simulink model "jumeau_banc_rw"  (R2025b)
settings: Solver=ode23t  StartTime=0.0  StopTime=20  MaxStep=1e-3  RelTol=1e-4
PostLoadFcn:
  | d = fileparts(get_param('jumeau_banc_rw', 'FileName')); addpath(fullfile(d, 'geometrie'), fullfile(d, 'liaison'), fullfile(d, 'pilotage')); clear d
StartFcn:
  | % Jumeau Webots : au lancement, MATLAB envoie les paramètres du Model Workspace à Webots, qui remet le banc en
  | % position de départ, puis ouvre la liaison de télémétrie et la liaison de commande (liaison/pont_banc.m).
  | if strcmp(get_param('jumeau_banc_rw/Procédé', 'LabelModeActiveChoice'), 'Webots')
  |     pont_banc('ouvrir', getVariable(get_param('jumeau_banc_rw', 'ModelWorkspace'), 'config_jumeau'));
  | end
  | pilotage_banc('depart');   % interface de pilotage : nouveau lancement
StopFcn:
  | pont_banc('fermer');
  | pilotage_banc('fin');
model workspace (MATLAB code in the model file):
  | %% Jumeau numérique du banc de stabilisation à 4 roues de réaction (version 3) : paramètres
  | % Ce code est enregistré dans le modèle (Model Explorer > jumeau_banc_rw > Model Workspace).
  | % Origine : (CAO) CAO du banc version 3, (M) mesuré sur le matériel, (F) fiche technique, (Fw) firmware,
  | % (H) hypothèse à mesurer sur le banc. Masses et inerties des pièces : dans chaque bloc de pièce.
  | 
  | %% Montage de l'essai
  | pivot_mm = 25;              % position du pivot de tangage sur le corps : 25, 24, 16, 8, 0, -8 mm (25 : banc équilibré, rangée +24 et paliers remontés de 1 mm)
  | blocage_roulis = 0;         % goupille de blocage : 1 = axe bloqué à 0°, 0 = axe libre
  | blocage_tangage = 0;
  | angle0_roulis_deg = 2;      % position de départ (mise à 0 si l'axe est bloqué)
  | angle0_tangage_deg = -1;
  | g = 9.81;                   % m/s²
  | 
  | %% Pupitre : pilotage manuel des 4 ESC
  | essai_t = 1;                % s, instant de l'échelon d'essai ajouté aux curseurs
  | essai_echelon_us = [0 0 0 0];   % µs, échelon d'essai sur chaque ESC (0 : aucun)
  | 
  | %% Alimentation des ESC
  | V_alim = 12;                % V, alimentation de labo (H : tension réglée)
  | 
  | %% ESC Brushless 30A bidirectionnels (x4)
  | f_trame_esc = 50;           % Hz, une impulsion toutes les 20 ms (Fw : LEDC 50 Hz)
  | imp_neutre = 1500;          % µs, neutre (testé sur le banc)
  | imp_min = 1000;             % µs (Fw)
  | imp_max = 2000;             % µs (Fw)
  | zone_morte_us = 0;          % µs autour du neutre (H)
  | tau_esc = 2e-3;             % s, temps de réponse de l'ESC (H)
  | armement_actif = 1;         % 1 : l'ESC ne pilote le moteur qu'après t_armement au neutre
  | t_armement = 1;             % s (H)
  | fenetre_armement_us = 25;   % µs, écart au neutre accepté pendant l'armement (H)
  | sens_moteurs = [1 1 1 1];   % +1 : au-dessus du neutre, la roue tourne dans le sens +axe (vers l'extérieur) (H : ordre des phases)
  | 
  | %% Moteurs A2212 1400 KV (x4), modèle équivalent continu
  | KV = 1400;                  % tr/min/V (F)
  | Ke = 60/(2*pi*KV);          % V.s/rad
  | Kt = Ke;                    % N.m/A
  | R_moteur = 0.08;            % ohm (H)
  | L_moteur = 30e-6;           % H (H)
  | f_roue = 5e-6;              % N.m.s/rad, frottement visqueux des roulements du moteur (H)
  | 
  | %% Cardan
  | butee_deg = 20;             % débattement de chaque axe (CAO)
  | k_butee = 20;               % N.m/rad, contact goupille-lumière (H)
  | c_butee = 0.2;              % N.m.s/rad (H)
  | b_cardan = 1e-4;            % N.m.s/rad, frottement des roulements 625 (H)
  | k_cables = 0;               % N.m/rad, raideur des deux câbles vers la table (H)
  | 
  | %% BNO055 (mode fusion)
  | T_bno = 0.01;               % s, données de fusion à 100 Hz (F)
  | bruit_bno = 1;              % 1 : bruit de mesure, 0 : capteur parfait
  | sigma_angle_deg = 0.05;     % ° (H)
  | sigma_gyro_dps = 0.1;       % °/s (H)
  | sigma_acc = 0.02;           % m/s² (H)
  | R_montage_bno = eye(3);     % axes du capteur dans le repère du dispositif : eye(3) = remappage AXIS_MAP réglé
  |                             % (la carte est tournée de 90° dans la CAO)
  | 
  | %% Capteurs de vitesse TCRT5000 (x4) : un front à chaque rayon du disque
  | n_rayons = 4;               % rayons du disque vus par tour (CAO : disque d'origine)
  | T_tcrt = 1e-3;              % s, pas de calcul du capteur (les fronts sont datés par interpolation, comme un chronomètre en µs)
  | t_arret_tcrt = 0.2;         % s sans front : la vitesse mesurée retombe à 0 (Fw, à fixer)
  | 
  | %% Pont vers le jumeau Webots (et, plus tard, vers l'ESP32 du banc réel)
  | T_pont = 0.01;              % s, une trame de commande et une trame de télémétrie toutes les 10 ms
  | 
  | %% Essai : maintien au départ et perturbation
  | t_lacher = 2;                % s, le dispositif est tenu à la main à sa position de départ jusqu'à cet instant (0 : libre dès le départ)
  | k_main = 5;                  % N.m/rad, raideur de la main qui tient le dispositif
  | c_main = 0.3;                % N.m.s/rad, son amortissement
  | perturbation_t = 7;          % s, instant de la poussée d'essai
  | perturbation_duree = 0.2;    % s
  | perturbation_couple = [0.02 0.02];   % N.m, couple de la poussée sur [roulis tangage], programmée (0 : aucune ; l'interface de pilotage en ajoute)
  | 
  | %% Grandeurs dérivées
  | assert(any(pivot_mm == [25 24 16 8 0 -8]), 'pivot_mm : 25, 24, 16, 8, 0, -8');
  | q0_deg = [angle0_roulis_deg angle0_tangage_deg] .* ([blocage_roulis blocage_tangage] == 0);
  | config_jumeau = [pivot_mm; blocage_roulis; blocage_tangage; q0_deg(:); V_alim; f_trame_esc; imp_neutre; imp_min; imp_max; ...
  |     zone_morte_us; tau_esc; armement_actif; t_armement; fenetre_armement_us; sens_moteurs(:); Ke; Kt; R_moteur; L_moteur; ...
  |     f_roue; butee_deg; k_butee; c_butee; b_cardan; k_cables; g; T_bno; bruit_bno; sigma_angle_deg; sigma_gyro_dps; ...
  |     sigma_acc; n_rayons; t_arret_tcrt; T_tcrt; R_montage_bno(:); T_pont; t_lacher; k_main; c_main];   % 51 valeurs envoyées au jumeau Webots au lancement
  | 
  | %% Commande bas niveau : une boucle de vitesse par roue, avec observateur CFO (méthode du TP2, ramenée à la vitesse)
  | J_roue = 1.562e-4;          % kg.m², inertie d'une roue autour de son axe : disque, vis, cloche du moteur (CAO)
  | T_cbn = 1/f_trame_esc;      % s, période de calcul de la commande : celle des ESC, qui ne lisent qu'une impulsion toutes les 20 ms
  | wc_roue = [10 10 10 10];    % rad/s, rapidité du suivi de vitesse de chaque roue (pôle de l'erreur en -wc)
  | wo_roue = [5 5 5 5];        % rad/s, rapidité du CFO de chaque roue (pôles en -wo et -4 wo) ; au-delà de 10, il devient instable à 20 ms
  | imp_cmd_min = 1375;         % µs, limites des impulsions commandées : vitesse conseillée des disques, 3 900 tr/min
  | imp_cmd_max = 1625;         % µs
  | w_aveugle = 45;             % rad/s, en dessous (vitesse du modèle), le TCRT5000 voit mal la roue : le CFO ne se corrige plus sur la mesure
  | 
  | %% Consigne d'essai des roues : ajoutée à la consigne qui vient de la conversion (0 tant qu'elle est vide)
  | essai_roue_t1 = 2;                  % s, départ vers le premier palier
  | essai_roue_vitesse1 = [0 0 0 0];  % rad/s, premier palier de chaque roue (0 : la roue reste à l'arrêt)
  | essai_roue_t2 = 6;                  % s, départ vers le second palier
  | essai_roue_vitesse2 = [0 0 0 0];    % rad/s, second palier de chaque roue
  | essai_roue_acc = 300;               % rad/s², pente des rampes entre les paliers
  | 
  | %% Commande bas niveau : grandeurs calculées
  | % modèle local d'une roue : d(omega)/dt = -a1 omega + a0 V + d
  | a0_roue = Kt/(R_moteur*J_roue) * [1 1 1 1];                % rad/s² par volt
  | a1_roue = (Kt*Ke/R_moteur + f_roue)/J_roue * [1 1 1 1];    % 1/s
  | K_roue = wc_roue - a1_roue;                                % retour d'état : erreur en -(a1 + K) = -wc
  | l1_roue = 5*wo_roue;                                       % CFO
  | lambda_roue = 4/5*wo_roue;
  | 
  | %% Référence : angles demandés au dispositif, en polynômes de degré 5 entre deux paliers
  | ref_t = [2 12];              % s, instant de départ vers chaque palier
  | ref_roulis_deg = [0 5];      % °, roulis demandé à chaque palier
  | ref_tangage_deg = [0 0];     % °, tangage demandé à chaque palier
  | ref_duree = 1.5;             % s, durée du passage d'un palier au suivant
  | 
  | %% Commande haut niveau : une boucle par axe [roulis tangage], placement de pôles basé sur l'observateur CFO (TP2)
  | T_chn = T_cbn;               % s, période de calcul : celle de la commande bas niveau et des ESC
  | t_depart = t_lacher;         % s, mise en marche de la commande : au moment où la main lâche le dispositif
  | wc_axe = [4 4];              % rad/s, rapidité du suivi d'angle de chaque axe
  | xi_axe = [1 1];              % amortissement
  | wo_axe = [3 3];              % rad/s, rapidité du CFO de chaque axe (pôles en -wo et -4 wo, double) ; au-delà de 4, le couple s'agite
  | desat_active = 0;            % 1 : la référence est décalée pour ramener les roues vers leur vitesse de repos
  | T_desat = 5;                 % s, constante de temps de ce retour
  | desat_max_deg = 15;          % °, décalage maximal de la référence
  | 
  | %% Conversion : couples des deux axes vers les 4 roues
  | w_repos = 200;               % rad/s, vitesse de repos des 4 roues : elles tournent toujours, le TCRT5000 les voit toujours
  | t_roues = t_armement + 0.2;  % s, mise en rotation des roues, une fois les ESC armés
  | acc_roue_max = 300;          % rad/s², accélération maximale demandée à une roue
  | w_roue_min = 60;             % rad/s, vitesses limites demandées à une roue
  | w_roue_max = 400;            % rad/s (disques : 3 900 tr/min conseillés, soit 408 rad/s)
  | 
  | %% Masses et inerties utilisées par la commande (CAO du banc version 3)
  | m_disp = 1.2615;             % kg, dispositif et ses 4 roues
  | zG_disp = 24.977e-3;         % m, hauteur de son centre de masse sur le corps (le pivot est à pivot_mm)
  | Ixx_disp_24 = 8.2684e-3;     % kg.m², inertie du dispositif autour du roulis, pivot à +24 mm
  | Iyy_disp_24 = 8.2786e-3;     % kg.m², autour du tangage, pivot à +24 mm
  | m_croix = 0.0755;            % kg, croisillon et paliers (ne tournent qu'en roulis)
  | zG_croix = 0.257e-3;         % m, hauteur de leur centre de masse au-dessus de l'axe de roulis
  | Ixx_croix = 2.073e-4;        % kg.m²
  | 
  | %% Commande haut niveau et conversion : grandeurs calculées
  | % modèle local d'un axe : d²(theta)/dt² = -a1 d(theta)/dt + a0 C + d, avec C le couple demandé aux roues
  | hz = zG_disp - pivot_mm/1000;                                    % m, centre de masse du dispositif au-dessus du pivot
  | I_axe = [Ixx_disp_24 + Ixx_croix, Iyy_disp_24] + m_disp*(hz^2 - (zG_disp - 0.024)^2) - 2*J_roue;   % kg.m²
  | mgh_axe = g*[m_disp*hz + m_croix*zG_croix, m_disp*hz];           % N.m/rad, couple de pesanteur par radian d'inclinaison
  | a0_axe = 1./I_axe;                                               % rad/s² par N.m
  | a1_axe = b_cardan./I_axe;                                        % 1/s
  | k1_axe = wc_axe.^2;                                              % retour d'état : s² + 2 xi wc s + wc²
  | k2_axe = 2*xi_axe.*wc_axe - a1_axe;
  | l1_axe = 9*wo_axe;                                               % CFO du TP2
  | l2_axe = 12*wo_axe.^2;
  | lambda_axe = 4/3*wo_axe;
  | C_max = 2*J_roue*cosd(45)*acc_roue_max;                          % N.m, couple maximal demandé sur un axe
  | k_desat = desat_active.*sign(mgh_axe + (mgh_axe == 0))./(max(abs(mgh_axe), 1e-3)*T_desat);            % rad par N.m.s
  | sx_roues = [1 -1 -1 1];                                          % signe de cos(45°, 135°, 225°, 315°) : part de chaque roue sur le roulis
  | sy_roues = [1 1 -1 -1];                                          % signe de sin : part sur le tangage
  | M_conv = -[sx_roues(:) sy_roues(:)]/(4*J_roue*cosd(45));         % accélération des 4 roues pour un couple [roulis; tangage]
  | 
  | %% Perception : des mesures à l'état du banc
  | T_perception = T_bno;        % s, période de calcul : celle du BNO055
  | tau_desequilibre = 2;        % s, constante de temps du filtre du couple extérieur et du déséquilibre
  | 
  | %% Pilotage par l'interface (pilotage/pilote_banc.m)
  | manche_max_deg = 15;         % °, limite de sécurité de l'inclinaison demandée par le manche (l'interface règle l'amplitude)
  | w_manche = 3;                % rad/s, rapidité avec laquelle la référence rejoint le manche (second ordre critique)
  | T_affichage = 0.1;           % s, rafraîchissement de l'interface
undefined symbols (not defined in the file): DiscIntNeverNeededParam, X, Y, Z
libraries: sm_lib x256, nesl_utility x24, simulink x7
(part 4 of 8)

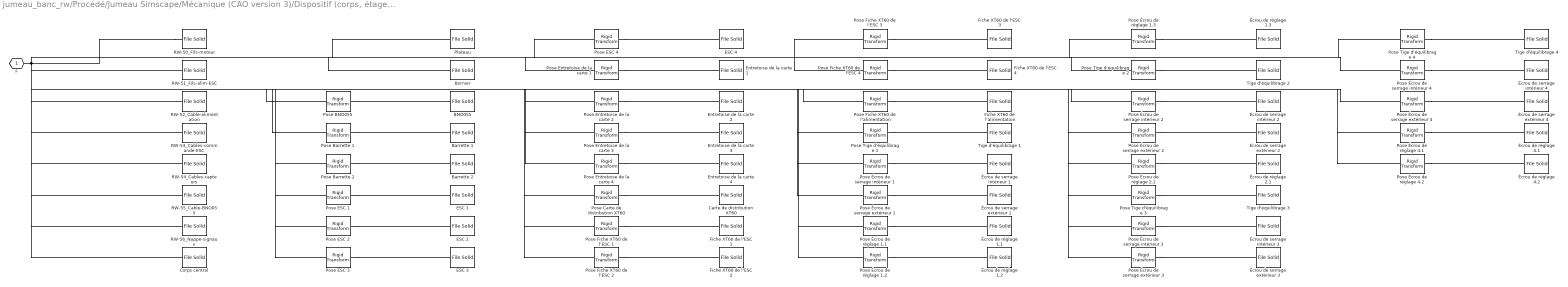
== system jumeau_banc_rw/Procédé/Jumeau Simscape/Mécanique (CAO version 3)/Dispositif (corps, étage, électronique, câblage) ==
  BNO055 : sm_lib/Body Elements/File Solid  Description=|  ExtGeomFileName=RW-32_BNO055.stl  UnitType=Custom  ExtGeomFileUnits=mm  StepReaderType=HEX  ExportConvexHullGeometry=off  InertiaType=Custom  BasedOnType=DensityFromFile  Density=1000  DensityUnits=kg/m^3  Mass=0.003  MassUnits=kg  CenterOfMass=[-2.1467412e-19 -0.0018514253 0.0013309763]  CenterOfMassUnits=m  MomentsOfInertia=[1.3564844e-07 1.7232429e-07 2.8762159e-07]  MomentsOfInertiaUnits=kg*m^2  ProductsOfInertia=[1.2064608e-08 -8.9985138e-25 -1.6417474e-24]  ProductsOfInertiaUnits=kg*m^2  GraphicType=FromGeometry  MarkerShape=Sphere  MarkerSize=10  GraphicVisPropType=SimpleVisualProperties  GraphicDiffuseColor=[0.173 0.627 0.173]  GraphicOpacity=1  GraphicSpecularColor=[0.5 0.5 0.5 1.0]  GraphicAmbientColor=[0.15 0.15 0.15 1.0]  GraphicEmissiveColor=[0.0 0.0 0.0 1.0]  GraphicShininess=75  DoExposeReferenceFrame=on  SerializedFrames=<Frames/>
      | Pièce CAO : BNO055 (RW-32_BNO055)
      | Masse 3.00 g : GY-BNO055, fiche, 3 g répartis sur le volume de la CAO.
      | Centre de masse et inertie : calculés sur la géométrie de la CAO.
  Barrette 1 : sm_lib/Body Elements/File Solid  Description=|  ExtGeomFileName=RW-36_Barrette-1x15.stl  UnitType=Custom  ExtGeomFileUnits=mm  StepReaderType=HEX  ExportConvexHullGeometry=off  InertiaType=Custom  BasedOnType=DensityFromFile  Density=1000  DensityUnits=kg/m^3  Mass=0.001  MassUnits=kg  CenterOfMass=[9.3534391e-19 3.3043458e-22 0.00027234952]  CenterOfMassUnits=m  MomentsOfInertia=[1.4288155e-08 1.347296e-07 1.2118031e-07]  MomentsOfInertiaUnits=kg*m^2  ProductsOfInertia=[-1.6381112e-26 2.6393535e-24 -2.0442735e-26]  ProductsOfInertiaUnits=kg*m^2  GraphicType=FromGeometry  MarkerShape=Sphere  MarkerSize=10  GraphicVisPropType=SimpleVisualProperties  GraphicDiffuseColor=[0.133 0.133 0.133]  GraphicOpacity=1  GraphicSpecularColor=[0.5 0.5 0.5 1.0]  GraphicAmbientColor=[0.15 0.15 0.15 1.0]  GraphicEmissiveColor=[0.0 0.0 0.0 1.0]  GraphicShininess=75  DoExposeReferenceFrame=on  SerializedFrames=<Frames/>
      | Pièce CAO : Barrette 1 (RW-36_Barrette-1x15)
      | Masse 1.00 g : barrette 1 × 15, estimée, 1 g répartis sur le volume de la CAO.
      | Centre de masse et inertie : calculés sur la géométrie de la CAO.
  Barrette 2 : sm_lib/Body Elements/File Solid  Description=|  ExtGeomFileName=RW-36_Barrette-1x15.stl  UnitType=Custom  ExtGeomFileUnits=mm  StepReaderType=HEX  ExportConvexHullGeometry=off  InertiaType=Custom  BasedOnType=DensityFromFile  Density=1000  DensityUnits=kg/m^3  Mass=0.001  MassUnits=kg  CenterOfMass=[9.3534391e-19 3.3043458e-22 0.00027234952]  CenterOfMassUnits=m  MomentsOfInertia=[1.4288155e-08 1.347296e-07 1.2118031e-07]  MomentsOfInertiaUnits=kg*m^2  ProductsOfInertia=[-1.6381112e-26 2.6393535e-24 -2.0442735e-26]  ProductsOfInertiaUnits=kg*m^2  GraphicType=FromGeometry  MarkerShape=Sphere  MarkerSize=10  GraphicVisPropType=SimpleVisualProperties  GraphicDiffuseColor=[0.133 0.133 0.133]  GraphicOpacity=1  GraphicSpecularColor=[0.5 0.5 0.5 1.0]  GraphicAmbientColor=[0.15 0.15 0.15 1.0]  GraphicEmissiveColor=[0.0 0.0 0.0 1.0]  GraphicShininess=75  DoExposeReferenceFrame=on  SerializedFrames=<Frames/>
      | Pièce CAO : Barrette 2 (RW-36_Barrette-1x15)
      | Masse 1.00 g : barrette 1 × 15, estimée, 1 g répartis sur le volume de la CAO.
      | Centre de masse et inertie : calculés sur la géométrie de la CAO.
  Bornier : sm_lib/Body Elements/File Solid  Description=|  ExtGeomFileName=RW-11_Bornier.stl  UnitType=Custom  ExtGeomFileUnits=mm  StepReaderType=HEX  ExportConvexHullGeometry=off  InertiaType=Custom  BasedOnType=DensityFromFile  Density=1000  DensityUnits=kg/m^3  Mass=0.0067119926  MassUnits=kg  CenterOfMass=[-0.07837267 3.6153019e-19 0.071437544]  CenterOfMassUnits=m  MomentsOfInertia=[1.208704e-06 5.2720754e-07 1.5981936e-06]  MomentsOfInertiaUnits=kg*m^2  ProductsOfInertia=[-5.3734654e-24 7.625406e-08 1.4773525e-23]  ProductsOfInertiaUnits=kg*m^2  GraphicType=FromGeometry  MarkerShape=Sphere  MarkerSize=10  GraphicVisPropType=SimpleVisualProperties  GraphicDiffuseColor=[0.867 0.518 0.322]  GraphicOpacity=1  GraphicSpecularColor=[0.5 0.5 0.5 1.0]  GraphicAmbientColor=[0.15 0.15 0.15 1.0]  GraphicEmissiveColor=[0.0 0.0 0.0 1.0]  GraphicShininess=75  DoExposeReferenceFrame=on  SerializedFrames=<Frames/>
      | Pièce CAO : Bornier (RW-11_Bornier)
      | Masse 6.71 g : PLA imprimé, 2 parois et 15 % de remplissage (hypothèse de conception), 800 kg/m³.
      | Centre de masse et inertie : calculés sur la géométrie de la CAO.
  Carte de distribution XT60 : sm_lib/Body Elements/File Solid  Description=|  ExtGeomFileName=RW-37_Carte-XT60-1x4.stl  UnitType=Custom  ExtGeomFileUnits=mm  StepReaderType=HEX  ExportConvexHullGeometry=off  InertiaType=Custom  BasedOnType=DensityFromFile  Density=1000  DensityUnits=kg/m^3  Mass=0.05  MassUnits=kg  CenterOfMass=[0.0081065575 2.9840954e-05 0.0051344044]  CenterOfMassUnits=m  MomentsOfInertia=[3.1408208e-06 3.157647e-05 3.2701875e-05]  MomentsOfInertiaUnits=kg*m^2  ProductsOfInertia=[2.2894046e-09 -1.2849535e-07 -3.2666061e-08]  ProductsOfInertiaUnits=kg*m^2  GraphicType=FromGeometry  MarkerShape=Sphere  MarkerSize=10  GraphicVisPropType=SimpleVisualProperties  GraphicDiffuseColor=[0.169 0.169 0.169]  GraphicOpacity=1  GraphicSpecularColor=[0.5 0.5 0.5 1.0]  GraphicAmbientColor=[0.15 0.15 0.15 1.0]  GraphicEmissiveColor=[0.0 0.0 0.0 1.0]  GraphicShininess=75  DoExposeReferenceFrame=on  SerializedFrames=<Frames/>
      | Pièce CAO : Carte de distribution XT60 (RW-37_Carte-XT60-1x4)
      | Masse 50.00 g : carte de distribution XT60 1 vers 4 (Jonronfey), estimée : carte 20 g, 4 embases 20 g, entrée 10 g, soit 50 g répartis sur le volume de la CAO.
      | Centre de masse et inertie : calculés sur la géométrie de la CAO.
  Corps central : sm_lib/Body Elements/File Solid  Description=|  ExtGeomFileName=RW-01_Moyeu.stl  UnitType=Custom  ExtGeomFileUnits=mm  StepReaderType=HEX  ExportConvexHullGeometry=off  InertiaType=Custom  BasedOnType=DensityFromFile  Density=1000  DensityUnits=kg/m^3  Mass=0.14444879  MassUnits=kg  CenterOfMass=[2.4874764e-15 1.1454189e-16 0.010858243]  CenterOfMassUnits=m  MomentsOfInertia=[0.00060979177 0.00056996624 0.000928403]  MomentsOfInertiaUnits=kg*m^2  ProductsOfInertia=[1.1230228e-19 -1.1420331e-17 -1.7396122e-07]  ProductsOfInertiaUnits=kg*m^2  GraphicType=FromGeometry  MarkerShape=Sphere  MarkerSize=10  GraphicVisPropType=SimpleVisualProperties  GraphicDiffuseColor=[0.298 0.447 0.69]  GraphicOpacity=1  GraphicSpecularColor=[0.5 0.5 0.5 1.0]  GraphicAmbientColor=[0.15 0.15 0.15 1.0]  GraphicEmissiveColor=[0.0 0.0 0.0 1.0]  GraphicShininess=75  DoExposeReferenceFrame=on  SerializedFrames=<Frames/>
      | Pièce CAO : Corps central (RW-01_Moyeu)
      | Masse 144.45 g : PLA imprimé, 2 parois et 15 % de remplissage (hypothèse de conception), 800 kg/m³.
      | Centre de masse et inertie : calculés sur la géométrie de la CAO.
  ESC 1 : sm_lib/Body Elements/File Solid  Description=|  ExtGeomFileName=RW-31_ESC-30A.stl  UnitType=Custom  ExtGeomFileUnits=mm  StepReaderType=HEX  ExportConvexHullGeometry=off  InertiaType=Custom  BasedOnType=DensityFromFile  Density=1000  DensityUnits=kg/m^3  Mass=0.028  MassUnits=kg  CenterOfMass=[-2.7359067e-19 2.5376526e-20 0.007]  CenterOfMassUnits=m  MomentsOfInertia=[2.8466667e-06 1.5390667e-05 1.7322667e-05]  MomentsOfInertiaUnits=kg*m^2  ProductsOfInertia=[0 3.8857806e-24 4.4408921e-24]  ProductsOfInertiaUnits=kg*m^2  GraphicType=FromGeometry  MarkerShape=Sphere  MarkerSize=10  GraphicVisPropType=SimpleVisualProperties  GraphicDiffuseColor=[0.506 0.447 0.702]  GraphicOpacity=1  GraphicSpecularColor=[0.5 0.5 0.5 1.0]  GraphicAmbientColor=[0.15 0.15 0.15 1.0]  GraphicEmissiveColor=[0.0 0.0 0.0 1.0]  GraphicShininess=75  DoExposeReferenceFrame=on  SerializedFrames=<Frames/>
      | Pièce CAO : ESC 1 (RW-31_ESC-30A)
      | Masse 28.00 g : ESC 30 A, fiche, 28 g répartis sur l'enveloppe de 80 × 32 × 14 mm.
      | Centre de masse et inertie : calculés sur la géométrie de la CAO.
  ESC 2 : sm_lib/Body Elements/File Solid  Description=|  ExtGeomFileName=RW-31_ESC-30A.stl  UnitType=Custom  ExtGeomFileUnits=mm  StepReaderType=HEX  ExportConvexHullGeometry=off  InertiaType=Custom  BasedOnType=DensityFromFile  Density=1000  DensityUnits=kg/m^3  Mass=0.028  MassUnits=kg  CenterOfMass=[-2.7359067e-19 2.5376526e-20 0.007]  CenterOfMassUnits=m  MomentsOfInertia=[2.8466667e-06 1.5390667e-05 1.7322667e-05]  MomentsOfInertiaUnits=kg*m^2  ProductsOfInertia=[0 3.8857806e-24 4.4408921e-24]  ProductsOfInertiaUnits=kg*m^2  GraphicType=FromGeometry  MarkerShape=Sphere  MarkerSize=10  GraphicVisPropType=SimpleVisualProperties  GraphicDiffuseColor=[0.506 0.447 0.702]  GraphicOpacity=1  GraphicSpecularColor=[0.5 0.5 0.5 1.0]  GraphicAmbientColor=[0.15 0.15 0.15 1.0]  GraphicEmissiveColor=[0.0 0.0 0.0 1.0]  GraphicShininess=75  DoExposeReferenceFrame=on  SerializedFrames=<Frames/>
      | Pièce CAO : ESC 2 (RW-31_ESC-30A)
      | Masse 28.00 g : ESC 30 A, fiche, 28 g répartis sur l'enveloppe de 80 × 32 × 14 mm.
      | Centre de masse et inertie : calculés sur la géométrie de la CAO.
  ESC 3 : sm_lib/Body Elements/File Solid  Description=|  ExtGeomFileName=RW-31_ESC-30A.stl  UnitType=Custom  ExtGeomFileUnits=mm  StepReaderType=HEX  ExportConvexHullGeometry=off  InertiaType=Custom  BasedOnType=DensityFromFile  Density=1000  DensityUnits=kg/m^3  Mass=0.028  MassUnits=kg  CenterOfMass=[-2.7359067e-19 2.5376526e-20 0.007]  CenterOfMassUnits=m  MomentsOfInertia=[2.8466667e-06 1.5390667e-05 1.7322667e-05]  MomentsOfInertiaUnits=kg*m^2  ProductsOfInertia=[0 3.8857806e-24 4.4408921e-24]  ProductsOfInertiaUnits=kg*m^2  GraphicType=FromGeometry  MarkerShape=Sphere  MarkerSize=10  GraphicVisPropType=SimpleVisualProperties  GraphicDiffuseColor=[0.506 0.447 0.702]  GraphicOpacity=1  GraphicSpecularColor=[0.5 0.5 0.5 1.0]  GraphicAmbientColor=[0.15 0.15 0.15 1.0]  GraphicEmissiveColor=[0.0 0.0 0.0 1.0]  GraphicShininess=75  DoExposeReferenceFrame=on  SerializedFrames=<Frames/>
      | Pièce CAO : ESC 3 (RW-31_ESC-30A)
      | Masse 28.00 g : ESC 30 A, fiche, 28 g répartis sur l'enveloppe de 80 × 32 × 14 mm.
      | Centre de masse et inertie : calculés sur la géométrie de la CAO.
  ESC 4 : sm_lib/Body Elements/File Solid  Description=|  ExtGeomFileName=RW-31_ESC-30A.stl  UnitType=Custom  ExtGeomFileUnits=mm  StepReaderType=HEX  ExportConvexHullGeometry=off  InertiaType=Custom  BasedOnType=DensityFromFile  Density=1000  DensityUnits=kg/m^3  Mass=0.028  MassUnits=kg  CenterOfMass=[-2.7359067e-19 2.5376526e-20 0.007]  CenterOfMassUnits=m  MomentsOfInertia=[2.8466667e-06 1.5390667e-05 1.7322667e-05]  MomentsOfInertiaUnits=kg*m^2  ProductsOfInertia=[0 3.8857806e-24 4.4408921e-24]  ProductsOfInertiaUnits=kg*m^2  GraphicType=FromGeometry  MarkerShape=Sphere  MarkerSize=10  GraphicVisPropType=SimpleVisualProperties  GraphicDiffuseColor=[0.506 0.447 0.702]  GraphicOpacity=1  GraphicSpecularColor=[0.5 0.5 0.5 1.0]  GraphicAmbientColor=[0.15 0.15 0.15 1.0]  GraphicEmissiveColor=[0.0 0.0 0.0 1.0]  GraphicShininess=75  DoExposeReferenceFrame=on  SerializedFrames=<Frames/>
      | Pièce CAO : ESC 4 (RW-31_ESC-30A)
      | Masse 28.00 g : ESC 30 A, fiche, 28 g répartis sur l'enveloppe de 80 × 32 × 14 mm.
      | Centre de masse et inertie : calculés sur la géométrie de la CAO.
  Entretoise de la carte 1 : sm_lib/Body Elements/File Solid  Description=|  ExtGeomFileName=RW-26_Entretoise-M3x35.stl  UnitType=Custom  ExtGeomFileUnits=mm  StepReaderType=HEX  ExportConvexHullGeometry=off  InertiaType=Custom  BasedOnType=DensityFromFile  Density=1000  DensityUnits=kg/m^3  Mass=0.0015  MassUnits=kg  CenterOfMass=[-3.7919292e-19 -1.1323077e-19 0.0175]  CenterOfMassUnits=m  MomentsOfInertia=[1.5749219e-07 1.5749219e-07 8.734375e-09]  MomentsOfInertiaUnits=kg*m^2  ProductsOfInertia=[1.2276244e-25 1.6949924e-24 5.0569321e-25]  ProductsOfInertiaUnits=kg*m^2  GraphicType=FromGeometry  MarkerShape=Sphere  MarkerSize=10  GraphicVisPropType=SimpleVisualProperties  GraphicDiffuseColor=[0.788 0.635 0.153]  GraphicOpacity=1  GraphicSpecularColor=[0.5 0.5 0.5 1.0]  GraphicAmbientColor=[0.15 0.15 0.15 1.0]  GraphicEmissiveColor=[0.0 0.0 0.0 1.0]  GraphicShininess=75  DoExposeReferenceFrame=on  SerializedFrames=<Frames/>
      | Pièce CAO : Entretoise de la carte 1 (RW-26_Entretoise-M3x35)
      | Masse 1.50 g : entretoise hexagonale M3 × 35, 1,5 g (nylon ; en laiton elle pèserait 6,3 g).
      | Centre de masse et inertie : calculés sur la géométrie de la CAO.
  Entretoise de la carte 2 : sm_lib/Body Elements/File Solid  Description=|  ExtGeomFileName=RW-26_Entretoise-M3x35.stl  UnitType=Custom  ExtGeomFileUnits=mm  StepReaderType=HEX  ExportConvexHullGeometry=off  InertiaType=Custom  BasedOnType=DensityFromFile  Density=1000  DensityUnits=kg/m^3  Mass=0.0015  MassUnits=kg  CenterOfMass=[-3.7919292e-19 -1.1323077e-19 0.0175]  CenterOfMassUnits=m  MomentsOfInertia=[1.5749219e-07 1.5749219e-07 8.734375e-09]  MomentsOfInertiaUnits=kg*m^2  ProductsOfInertia=[1.2276244e-25 1.6949924e-24 5.0569321e-25]  ProductsOfInertiaUnits=kg*m^2  GraphicType=FromGeometry  MarkerShape=Sphere  MarkerSize=10  GraphicVisPropType=SimpleVisualProperties  GraphicDiffuseColor=[0.788 0.635 0.153]  GraphicOpacity=1  GraphicSpecularColor=[0.5 0.5 0.5 1.0]  GraphicAmbientColor=[0.15 0.15 0.15 1.0]  GraphicEmissiveColor=[0.0 0.0 0.0 1.0]  GraphicShininess=75  DoExposeReferenceFrame=on  SerializedFrames=<Frames/>
      | Pièce CAO : Entretoise de la carte 2 (RW-26_Entretoise-M3x35)
      | Masse 1.50 g : entretoise hexagonale M3 × 35, 1,5 g (nylon ; en laiton elle pèserait 6,3 g).
      | Centre de masse et inertie : calculés sur la géométrie de la CAO.
  Entretoise de la carte 3 : sm_lib/Body Elements/File Solid  Description=|  ExtGeomFileName=RW-26_Entretoise-M3x35.stl  UnitType=Custom  ExtGeomFileUnits=mm  StepReaderType=HEX  ExportConvexHullGeometry=off  InertiaType=Custom  BasedOnType=DensityFromFile  Density=1000  DensityUnits=kg/m^3  Mass=0.0015  MassUnits=kg  CenterOfMass=[-3.7919292e-19 -1.1323077e-19 0.0175]  CenterOfMassUnits=m  MomentsOfInertia=[1.5749219e-07 1.5749219e-07 8.734375e-09]  MomentsOfInertiaUnits=kg*m^2  ProductsOfInertia=[1.2276244e-25 1.6949924e-24 5.0569321e-25]  ProductsOfInertiaUnits=kg*m^2  GraphicType=FromGeometry  MarkerShape=Sphere  MarkerSize=10  GraphicVisPropType=SimpleVisualProperties  GraphicDiffuseColor=[0.788 0.635 0.153]  GraphicOpacity=1  GraphicSpecularColor=[0.5 0.5 0.5 1.0]  GraphicAmbientColor=[0.15 0.15 0.15 1.0]  GraphicEmissiveColor=[0.0 0.0 0.0 1.0]  GraphicShininess=75  DoExposeReferenceFrame=on  SerializedFrames=<Frames/>
      | Pièce CAO : Entretoise de la carte 3 (RW-26_Entretoise-M3x35)
      | Masse 1.50 g : entretoise hexagonale M3 × 35, 1,5 g (nylon ; en laiton elle pèserait 6,3 g).
      | Centre de masse et inertie : calculés sur la géométrie de la CAO.
  Entretoise de la carte 4 : sm_lib/Body Elements/File Solid  Description=|  ExtGeomFileName=RW-26_Entretoise-M3x35.stl  UnitType=Custom  ExtGeomFileUnits=mm  StepReaderType=HEX  ExportConvexHullGeometry=off  InertiaType=Custom  BasedOnType=DensityFromFile  Density=1000  DensityUnits=kg/m^3  Mass=0.0015  MassUnits=kg  CenterOfMass=[-3.7919292e-19 -1.1323077e-19 0.0175]  CenterOfMassUnits=m  MomentsOfInertia=[1.5749219e-07 1.5749219e-07 8.734375e-09]  MomentsOfInertiaUnits=kg*m^2  ProductsOfInertia=[1.2276244e-25 1.6949924e-24 5.0569321e-25]  ProductsOfInertiaUnits=kg*m^2  GraphicType=FromGeometry  MarkerShape=Sphere  MarkerSize=10  GraphicVisPropType=SimpleVisualProperties  GraphicDiffuseColor=[0.788 0.635 0.153]  GraphicOpacity=1  GraphicSpecularColor=[0.5 0.5 0.5 1.0]  GraphicAmbientColor=[0.15 0.15 0.15 1.0]  GraphicEmissiveColor=[0.0 0.0 0.0 1.0]  GraphicShininess=75  DoExposeReferenceFrame=on  SerializedFrames=<Frames/>
      | Pièce CAO : Entretoise de la carte 4 (RW-26_Entretoise-M3x35)
      | Masse 1.50 g : entretoise hexagonale M3 × 35, 1,5 g (nylon ; en laiton elle pèserait 6,3 g).
      | Centre de masse et inertie : calculés sur la géométrie de la CAO.
  Fiche XT60 de l'ESC 1 : sm_lib/Body Elements/File Solid  Description=|  ExtGeomFileName=RW-38_Fiche-XT60.stl  UnitType=Custom  ExtGeomFileUnits=mm  StepReaderType=HEX  ExportConvexHullGeometry=off  InertiaType=Custom  BasedOnType=DensityFromFile  Density=1000  DensityUnits=kg/m^3  Mass=0.005  MassUnits=kg  CenterOfMass=[-2.9282725e-20 1.5143192e-19 0.006]  CenterOfMassUnits=m  MomentsOfInertia=[1.614e-07 8.8016667e-08 1.2941667e-07]  MomentsOfInertiaUnits=kg*m^2  ProductsOfInertia=[4.4436694e-24 5.3376107e-26 -1.1564823e-26]  ProductsOfInertiaUnits=kg*m^2  GraphicType=FromGeometry  MarkerShape=Sphere  MarkerSize=10  GraphicVisPropType=SimpleVisualProperties  GraphicDiffuseColor=[0.91 0.773 0.278]  GraphicOpacity=1  GraphicSpecularColor=[0.5 0.5 0.5 1.0]  GraphicAmbientColor=[0.15 0.15 0.15 1.0]  GraphicEmissiveColor=[0.0 0.0 0.0 1.0]  GraphicShininess=75  DoExposeReferenceFrame=on  SerializedFrames=<Frames/>
      | Pièce CAO : Fiche XT60 de l'ESC 1 (RW-38_Fiche-XT60)
      | Masse 5.00 g : fiche XT60 d'un ESC, estimée, 5 g.
      | Centre de masse et inertie : calculés sur la géométrie de la CAO.
  Fiche XT60 de l'ESC 2 : sm_lib/Body Elements/File Solid  Description=|  ExtGeomFileName=RW-38_Fiche-XT60.stl  UnitType=Custom  ExtGeomFileUnits=mm  StepReaderType=HEX  ExportConvexHullGeometry=off  InertiaType=Custom  BasedOnType=DensityFromFile  Density=1000  DensityUnits=kg/m^3  Mass=0.005  MassUnits=kg  CenterOfMass=[-2.9282725e-20 1.5143192e-19 0.006]  CenterOfMassUnits=m  MomentsOfInertia=[1.614e-07 8.8016667e-08 1.2941667e-07]  MomentsOfInertiaUnits=kg*m^2  ProductsOfInertia=[4.4436694e-24 5.3376107e-26 -1.1564823e-26]  ProductsOfInertiaUnits=kg*m^2  GraphicType=FromGeometry  MarkerShape=Sphere  MarkerSize=10  GraphicVisPropType=SimpleVisualProperties  GraphicDiffuseColor=[0.91 0.773 0.278]  GraphicOpacity=1  GraphicSpecularColor=[0.5 0.5 0.5 1.0]  GraphicAmbientColor=[0.15 0.15 0.15 1.0]  GraphicEmissiveColor=[0.0 0.0 0.0 1.0]  GraphicShininess=75  DoExposeReferenceFrame=on  SerializedFrames=<Frames/>
      | Pièce CAO : Fiche XT60 de l'ESC 2 (RW-38_Fiche-XT60)
      | Masse 5.00 g : fiche XT60 d'un ESC, estimée, 5 g.
      | Centre de masse et inertie : calculés sur la géométrie de la CAO.
  Fiche XT60 de l'ESC 3 : sm_lib/Body Elements/File Solid  Description=|  ExtGeomFileName=RW-38_Fiche-XT60.stl  UnitType=Custom  ExtGeomFileUnits=mm  StepReaderType=HEX  ExportConvexHullGeometry=off  InertiaType=Custom  BasedOnType=DensityFromFile  Density=1000  DensityUnits=kg/m^3  Mass=0.005  MassUnits=kg  CenterOfMass=[-2.9282725e-20 1.5143192e-19 0.006]  CenterOfMassUnits=m  MomentsOfInertia=[1.614e-07 8.8016667e-08 1.2941667e-07]  MomentsOfInertiaUnits=kg*m^2  ProductsOfInertia=[4.4436694e-24 5.3376107e-26 -1.1564823e-26]  ProductsOfInertiaUnits=kg*m^2  GraphicType=FromGeometry  MarkerShape=Sphere  MarkerSize=10  GraphicVisPropType=SimpleVisualProperties  GraphicDiffuseColor=[0.91 0.773 0.278]  GraphicOpacity=1  GraphicSpecularColor=[0.5 0.5 0.5 1.0]  GraphicAmbientColor=[0.15 0.15 0.15 1.0]  GraphicEmissiveColor=[0.0 0.0 0.0 1.0]  GraphicShininess=75  DoExposeReferenceFrame=on  SerializedFrames=<Frames/>
      | Pièce CAO : Fiche XT60 de l'ESC 3 (RW-38_Fiche-XT60)
      | Masse 5.00 g : fiche XT60 d'un ESC, estimée, 5 g.
      | Centre de masse et inertie : calculés sur la géométrie de la CAO.
  Fiche XT60 de l'ESC 4 : sm_lib/Body Elements/File Solid  Description=|  ExtGeomFileName=RW-38_Fiche-XT60.stl  UnitType=Custom  ExtGeomFileUnits=mm  StepReaderType=HEX  ExportConvexHullGeometry=off  InertiaType=Custom  BasedOnType=DensityFromFile  Density=1000  DensityUnits=kg/m^3  Mass=0.005  MassUnits=kg  CenterOfMass=[-2.9282725e-20 1.5143192e-19 0.006]  CenterOfMassUnits=m  MomentsOfInertia=[1.614e-07 8.8016667e-08 1.2941667e-07]  MomentsOfInertiaUnits=kg*m^2  ProductsOfInertia=[4.4436694e-24 5.3376107e-26 -1.1564823e-26]  ProductsOfInertiaUnits=kg*m^2  GraphicType=FromGeometry  MarkerShape=Sphere  MarkerSize=10  GraphicVisPropType=SimpleVisualProperties  GraphicDiffuseColor=[0.91 0.773 0.278]  GraphicOpacity=1  GraphicSpecularColor=[0.5 0.5 0.5 1.0]  GraphicAmbientColor=[0.15 0.15 0.15 1.0]  GraphicEmissiveColor=[0.0 0.0 0.0 1.0]  GraphicShininess=75  DoExposeReferenceFrame=on  SerializedFrames=<Frames/>
      | Pièce CAO : Fiche XT60 de l'ESC 4 (RW-38_Fiche-XT60)
      | Masse 5.00 g : fiche XT60 d'un ESC, estimée, 5 g.
      | Centre de masse et inertie : calculés sur la géométrie de la CAO.
  Fiche XT60 de l'alimentation : sm_lib/Body Elements/File Solid  Description=|  ExtGeomFileName=RW-39_Fiche-XT60-alim.stl  UnitType=Custom  ExtGeomFileUnits=mm  StepReaderType=HEX  ExportConvexHullGeometry=off  InertiaType=Custom  BasedOnType=DensityFromFile  Density=1000  DensityUnits=kg/m^3  Mass=0.005  MassUnits=kg  CenterOfMass=[-2.1784124e-20 -1.4742799e-20 0.008]  CenterOfMassUnits=m  MomentsOfInertia=[2.0806667e-07 1.3468333e-07 1.2941667e-07]  MomentsOfInertiaUnits=kg*m^2  ProductsOfInertia=[-2.466732e-40 -8.8960178e-27 -2.6020852e-26]  ProductsOfInertiaUnits=kg*m^2  GraphicType=FromGeometry  MarkerShape=Sphere  MarkerSize=10  GraphicVisPropType=SimpleVisualProperties  GraphicDiffuseColor=[0.91 0.773 0.278]  GraphicOpacity=1  GraphicSpecularColor=[0.5 0.5 0.5 1.0]  GraphicAmbientColor=[0.15 0.15 0.15 1.0]  GraphicEmissiveColor=[0.0 0.0 0.0 1.0]  GraphicShininess=75  DoExposeReferenceFrame=on  SerializedFrames=<Frames/>
      | Pièce CAO : Fiche XT60 de l'alimentation (RW-39_Fiche-XT60-alim)
      | Masse 5.00 g : fiche XT60 du câble d'alimentation, estimée, 5 g.
      | Centre de masse et inertie : calculés sur la géométrie de la CAO.
  Plateau : sm_lib/Body Elements/File Solid  Description=|  ExtGeomFileName=RW-08_Plateau.stl  UnitType=Custom  ExtGeomFileUnits=mm  StepReaderType=HEX  ExportConvexHullGeometry=off  InertiaType=Custom  BasedOnType=DensityFromFile  Density=1000  DensityUnits=kg/m^3  Mass=0.08982138  MassUnits=kg  CenterOfMass=[7.5433571e-05 3.5587293e-05 0.064259887]  CenterOfMassUnits=m  MomentsOfInertia=[0.00015384632 0.00015355924 0.00030323992]  MomentsOfInertiaUnits=kg*m^2  ProductsOfInertia=[5.0443796e-09 1.2680935e-08 -4.9020861e-09]  ProductsOfInertiaUnits=kg*m^2  GraphicType=FromGeometry  MarkerShape=Sphere  MarkerSize=10  GraphicVisPropType=SimpleVisualProperties  GraphicDiffuseColor=[0.416 0.561 0.784]  GraphicOpacity=1  GraphicSpecularColor=[0.5 0.5 0.5 1.0]  GraphicAmbientColor=[0.15 0.15 0.15 1.0]  GraphicEmissiveColor=[0.0 0.0 0.0 1.0]  GraphicShininess=75  DoExposeReferenceFrame=on  SerializedFrames=<Frames/>
      | Pièce CAO : Plateau (RW-08_Plateau)
      | Masse 89.82 g : PLA imprimé, 2 parois et 15 % de remplissage (hypothèse de conception), 800 kg/m³.
      | Centre de masse et inertie : calculés sur la géométrie de la CAO.
  Pose BNO055 : sm_lib/Frames and Transforms/Rigid Transform  RotationMethod=RotationMatrix  FollAlignAxisA=+X  BaseAlignAxisA=+Y  FollAlignAxisB=+Y  BaseAlignAxisB=+Z  RotationStandardAxis=+Z  RotationAngle=0  RotationAngleUnits=deg  RotationArbitraryAxis=[0 0 1]  RotationSequenceAxes=FollowerAxes  RotationSequence=XYX  RotationSequenceAngles=[0 0 0]  RotationSequenceAnglesUnits=deg  RotationMatrix=[0 1 0;-1 0 0;0 0 1]  Quaternion=[1 0 0 0]  TranslationMethod=Cartesian  TranslationCartesianOffset=[0 0 64]  TranslationCartesianOffsetUnits=mm  TranslationStandardAxis=+Z  TranslationStandardOffset=0  TranslationStandardOffsetUnits=m  TranslationROffset=0  TranslationROffsetUnits=m  TranslationThetaOffset=0  TranslationThetaOffsetUnits=deg  TranslationZOffset=0  TranslationZOffsetUnits=m
  Pose Barrette 1 : sm_lib/Frames and Transforms/Rigid Transform  RotationMethod=RotationMatrix  FollAlignAxisA=+X  BaseAlignAxisA=+Y  FollAlignAxisB=+Y  BaseAlignAxisB=+Z  RotationStandardAxis=+Z  RotationAngle=0  RotationAngleUnits=deg  RotationArbitraryAxis=[0 0 1]  RotationSequenceAxes=FollowerAxes  RotationSequence=XYX  RotationSequenceAngles=[0 0 0]  RotationSequenceAnglesUnits=deg  RotationMatrix=[0 -1 0;1 0 0;0 0 1]  Quaternion=[1 0 0 0]  TranslationMethod=Cartesian  TranslationCartesianOffset=[-85 0 73.4]  TranslationCartesianOffsetUnits=mm  TranslationStandardAxis=+Z  TranslationStandardOffset=0  TranslationStandardOffsetUnits=m  TranslationROffset=0  TranslationROffsetUnits=m  TranslationThetaOffset=0  TranslationThetaOffsetUnits=deg  TranslationZOffset=0  TranslationZOffsetUnits=m
  Pose Barrette 2 : sm_lib/Frames and Transforms/Rigid Transform  RotationMethod=RotationMatrix  FollAlignAxisA=+X  BaseAlignAxisA=+Y  FollAlignAxisB=+Y  BaseAlignAxisB=+Z  RotationStandardAxis=+Z  RotationAngle=0  RotationAngleUnits=deg  RotationArbitraryAxis=[0 0 1]  RotationSequenceAxes=FollowerAxes  RotationSequence=XYX  RotationSequenceAngles=[0 0 0]  RotationSequenceAnglesUnits=deg  RotationMatrix=[0 -1 0;1 0 0;0 0 1]  Quaternion=[1 0 0 0]  TranslationMethod=Cartesian  TranslationCartesianOffset=[-91 0 73.4]  TranslationCartesianOffsetUnits=mm  TranslationStandardAxis=+Z  TranslationStandardOffset=0  TranslationStandardOffsetUnits=m  TranslationROffset=0  TranslationROffsetUnits=m  TranslationThetaOffset=0  TranslationThetaOffsetUnits=deg  TranslationZOffset=0  TranslationZOffsetUnits=m
  Pose Carte de distribution XT60 : sm_lib/Frames and Transforms/Rigid Transform  RotationMethod=RotationMatrix  FollAlignAxisA=+X  BaseAlignAxisA=+Y  FollAlignAxisB=+Y  BaseAlignAxisB=+Z  RotationStandardAxis=+Z  RotationAngle=0  RotationAngleUnits=deg  RotationArbitraryAxis=[0 0 1]  RotationSequenceAxes=FollowerAxes  RotationSequence=XYX  RotationSequenceAngles=[0 0 0]  RotationSequenceAnglesUnits=deg  RotationMatrix=[1 0 0;0 1 0;0 0 1]  Quaternion=[1 0 0 0]  TranslationMethod=Cartesian  TranslationCartesianOffset=[0 0 100]  TranslationCartesianOffsetUnits=mm  TranslationStandardAxis=+Z  TranslationStandardOffset=0  TranslationStandardOffsetUnits=m  TranslationROffset=0  TranslationROffsetUnits=m  TranslationThetaOffset=0  TranslationThetaOffsetUnits=deg  TranslationZOffset=0  TranslationZOffsetUnits=m
  Pose ESC 1 : sm_lib/Frames and Transforms/Rigid Transform  RotationMethod=RotationMatrix  FollAlignAxisA=+X  BaseAlignAxisA=+Y  FollAlignAxisB=+Y  BaseAlignAxisB=+Z  RotationStandardAxis=+Z  RotationAngle=0  RotationAngleUnits=deg  RotationArbitraryAxis=[0 0 1]  RotationSequenceAxes=FollowerAxes  RotationSequence=XYX  RotationSequenceAngles=[0 0 0]  RotationSequenceAnglesUnits=deg  RotationMatrix=[0 0 1;1 0 0;0 1 0]  Quaternion=[1 0 0 0]  TranslationMethod=Cartesian  TranslationCartesianOffset=[46 0 81]  TranslationCartesianOffsetUnits=mm  TranslationStandardAxis=+Z  TranslationStandardOffset=0  TranslationStandardOffsetUnits=m  TranslationROffset=0  TranslationROffsetUnits=m  TranslationThetaOffset=0  TranslationThetaOffsetUnits=deg  TranslationZOffset=0  TranslationZOffsetUnits=m
  Pose ESC 2 : sm_lib/Frames and Transforms/Rigid Transform  RotationMethod=RotationMatrix  FollAlignAxisA=+X  BaseAlignAxisA=+Y  FollAlignAxisB=+Y  BaseAlignAxisB=+Z  RotationStandardAxis=+Z  RotationAngle=0  RotationAngleUnits=deg  RotationArbitraryAxis=[0 0 1]  RotationSequenceAxes=FollowerAxes  RotationSequence=XYX  RotationSequenceAngles=[0 0 0]  RotationSequenceAnglesUnits=deg  RotationMatrix=[-1 0 0;0 0 1;0 1 0]  Quaternion=[1 0 0 0]  TranslationMethod=Cartesian  TranslationCartesianOffset=[0 46 81]  TranslationCartesianOffsetUnits=mm  TranslationStandardAxis=+Z  TranslationStandardOffset=0  TranslationStandardOffsetUnits=m  TranslationROffset=0  TranslationROffsetUnits=m  TranslationThetaOffset=0  TranslationThetaOffsetUnits=deg  TranslationZOffset=0  TranslationZOffsetUnits=m
  Pose ESC 3 : sm_lib/Frames and Transforms/Rigid Transform  RotationMethod=RotationMatrix  FollAlignAxisA=+X  BaseAlignAxisA=+Y  FollAlignAxisB=+Y  BaseAlignAxisB=+Z  RotationStandardAxis=+Z  RotationAngle=0  RotationAngleUnits=deg  RotationArbitraryAxis=[0 0 1]  RotationSequenceAxes=FollowerAxes  RotationSequence=XYX  RotationSequenceAngles=[0 0 0]  RotationSequenceAnglesUnits=deg  RotationMatrix=[0 0 -1;-1 0 0;0 1 0]  Quaternion=[1 0 0 0]  TranslationMethod=Cartesian  TranslationCartesianOffset=[-46 0 81]  TranslationCartesianOffsetUnits=mm  TranslationStandardAxis=+Z  TranslationStandardOffset=0  TranslationStandardOffsetUnits=m  TranslationROffset=0  TranslationROffsetUnits=m  TranslationThetaOffset=0  TranslationThetaOffsetUnits=deg  TranslationZOffset=0  TranslationZOffsetUnits=m
  Pose ESC 4 : sm_lib/Frames and Transforms/Rigid Transform  RotationMethod=RotationMatrix  FollAlignAxisA=+X  BaseAlignAxisA=+Y  FollAlignAxisB=+Y  BaseAlignAxisB=+Z  RotationStandardAxis=+Z  RotationAngle=0  RotationAngleUnits=deg  RotationArbitraryAxis=[0 0 1]  RotationSequenceAxes=FollowerAxes  RotationSequence=XYX  RotationSequenceAngles=[0 0 0]  RotationSequenceAnglesUnits=deg  RotationMatrix=[1 0 0;0 0 -1;0 1 0]  Quaternion=[1 0 0 0]  TranslationMethod=Cartesian  TranslationCartesianOffset=[0 -46 81]  TranslationCartesianOffsetUnits=mm  TranslationStandardAxis=+Z  TranslationStandardOffset=0  TranslationStandardOffsetUnits=m  TranslationROffset=0  TranslationROffsetUnits=m  TranslationThetaOffset=0  TranslationThetaOffsetUnits=deg  TranslationZOffset=0  TranslationZOffsetUnits=m
  Pose Entretoise de la carte 1 : sm_lib/Frames and Transforms/Rigid Transform  RotationMethod=RotationMatrix  FollAlignAxisA=+X  BaseAlignAxisA=+Y  FollAlignAxisB=+Y  BaseAlignAxisB=+Z  RotationStandardAxis=+Z  RotationAngle=0  RotationAngleUnits=deg  RotationArbitraryAxis=[0 0 1]  RotationSequenceAxes=FollowerAxes  RotationSequence=XYX  RotationSequenceAngles=[0 0 0]  RotationSequenceAnglesUnits=deg  RotationMatrix=[1 0 0;0 1 0;0 0 1]  Quaternion=[1 0 0 0]  TranslationMethod=Cartesian  TranslationCartesianOffset=[-33 -12 65]  TranslationCartesianOffsetUnits=mm  TranslationStandardAxis=+Z  TranslationStandardOffset=0  TranslationStandardOffsetUnits=m  TranslationROffset=0  TranslationROffsetUnits=m  TranslationThetaOffset=0  TranslationThetaOffsetUnits=deg  TranslationZOffset=0  TranslationZOffsetUnits=m
  Pose Entretoise de la carte 2 : sm_lib/Frames and Transforms/Rigid Transform  RotationMethod=RotationMatrix  FollAlignAxisA=+X  BaseAlignAxisA=+Y  FollAlignAxisB=+Y  BaseAlignAxisB=+Z  RotationStandardAxis=+Z  RotationAngle=0  RotationAngleUnits=deg  RotationArbitraryAxis=[0 0 1]  RotationSequenceAxes=FollowerAxes  RotationSequence=XYX  RotationSequenceAngles=[0 0 0]  RotationSequenceAnglesUnits=deg  RotationMatrix=[1 0 0;0 1 0;0 0 1]  Quaternion=[1 0 0 0]  TranslationMethod=Cartesian  TranslationCartesianOffset=[-33 12 65]  TranslationCartesianOffsetUnits=mm  TranslationStandardAxis=+Z  TranslationStandardOffset=0  TranslationStandardOffsetUnits=m  TranslationROffset=0  TranslationROffsetUnits=m  TranslationThetaOffset=0  TranslationThetaOffsetUnits=deg  TranslationZOffset=0  TranslationZOffsetUnits=m
  Pose Entretoise de la carte 3 : sm_lib/Frames and Transforms/Rigid Transform  RotationMethod=RotationMatrix  FollAlignAxisA=+X  BaseAlignAxisA=+Y  FollAlignAxisB=+Y  BaseAlignAxisB=+Z  RotationStandardAxis=+Z  RotationAngle=0  RotationAngleUnits=deg  RotationArbitraryAxis=[0 0 1]  RotationSequenceAxes=FollowerAxes  RotationSequence=XYX  RotationSequenceAngles=[0 0 0]  RotationSequenceAnglesUnits=deg  RotationMatrix=[1 0 0;0 1 0;0 0 1]  Quaternion=[1 0 0 0]  TranslationMethod=Cartesian  TranslationCartesianOffset=[33 -12 65]  TranslationCartesianOffsetUnits=mm  TranslationStandardAxis=+Z  TranslationStandardOffset=0  TranslationStandardOffsetUnits=m  TranslationROffset=0  TranslationROffsetUnits=m  TranslationThetaOffset=0  TranslationThetaOffsetUnits=deg  TranslationZOffset=0  TranslationZOffsetUnits=m
  Pose Entretoise de la carte 4 : sm_lib/Frames and Transforms/Rigid Transform  RotationMethod=RotationMatrix  FollAlignAxisA=+X  BaseAlignAxisA=+Y  FollAlignAxisB=+Y  BaseAlignAxisB=+Z  RotationStandardAxis=+Z  RotationAngle=0  RotationAngleUnits=deg  RotationArbitraryAxis=[0 0 1]  RotationSequenceAxes=FollowerAxes  RotationSequence=XYX  RotationSequenceAngles=[0 0 0]  RotationSequenceAnglesUnits=deg  RotationMatrix=[1 0 0;0 1 0;0 0 1]  Quaternion=[1 0 0 0]  TranslationMethod=Cartesian  TranslationCartesianOffset=[33 12 65]  TranslationCartesianOffsetUnits=mm  TranslationStandardAxis=+Z  TranslationStandardOffset=0  TranslationStandardOffsetUnits=m  TranslationROffset=0  TranslationROffsetUnits=m  TranslationThetaOffset=0  TranslationThetaOffsetUnits=deg  TranslationZOffset=0  TranslationZOffsetUnits=m
  Pose Fiche XT60 de l'ESC 1 : sm_lib/Frames and Transforms/Rigid Transform  RotationMethod=RotationMatrix  FollAlignAxisA=+X  BaseAlignAxisA=+Y  FollAlignAxisB=+Y  BaseAlignAxisB=+Z  RotationStandardAxis=+Z  RotationAngle=0  RotationAngleUnits=deg  RotationArbitraryAxis=[0 0 1]  RotationSequenceAxes=FollowerAxes  RotationSequence=XYX  RotationSequenceAngles=[0 0 0]  RotationSequenceAnglesUnits=deg  RotationMatrix=[1 0 0;0 1 0;0 0 1]  Quaternion=[1 0 0 0]  TranslationMethod=Cartesian  TranslationCartesianOffset=[1.3 0 117.6]  TranslationCartesianOffsetUnits=mm  TranslationStandardAxis=+Z  TranslationStandardOffset=0  TranslationStandardOffsetUnits=m  TranslationROffset=0  TranslationROffsetUnits=m  TranslationThetaOffset=0  TranslationThetaOffsetUnits=deg  TranslationZOffset=0  TranslationZOffsetUnits=m
  Pose Fiche XT60 de l'ESC 2 : sm_lib/Frames and Transforms/Rigid Transform  RotationMethod=RotationMatrix  FollAlignAxisA=+X  BaseAlignAxisA=+Y  FollAlignAxisB=+Y  BaseAlignAxisB=+Z  RotationStandardAxis=+Z  RotationAngle=0  RotationAngleUnits=deg  RotationArbitraryAxis=[0 0 1]  RotationSequenceAxes=FollowerAxes  RotationSequence=XYX  RotationSequenceAngles=[0 0 0]  RotationSequenceAnglesUnits=deg  RotationMatrix=[1 0 0;0 1 0;0 0 1]  Quaternion=[1 0 0 0]  TranslationMethod=Cartesian  TranslationCartesianOffset=[15.3 0 117.6]  TranslationCartesianOffsetUnits=mm  TranslationStandardAxis=+Z  TranslationStandardOffset=0  TranslationStandardOffsetUnits=m  TranslationROffset=0  TranslationROffsetUnits=m  TranslationThetaOffset=0  TranslationThetaOffsetUnits=deg  TranslationZOffset=0  TranslationZOffsetUnits=m
  Pose Fiche XT60 de l'ESC 3 : sm_lib/Frames and Transforms/Rigid Transform  RotationMethod=RotationMatrix  FollAlignAxisA=+X  BaseAlignAxisA=+Y  FollAlignAxisB=+Y  BaseAlignAxisB=+Z  RotationStandardAxis=+Z  RotationAngle=0  RotationAngleUnits=deg  RotationArbitraryAxis=[0 0 1]  RotationSequenceAxes=FollowerAxes  RotationSequence=XYX  RotationSequenceAngles=[0 0 0]  RotationSequenceAnglesUnits=deg  RotationMatrix=[1 0 0;0 1 0;0 0 1]  Quaternion=[1 0 0 0]  TranslationMethod=Cartesian  TranslationCartesianOffset=[-14.8 0 117.6]  TranslationCartesianOffsetUnits=mm  TranslationStandardAxis=+Z  TranslationStandardOffset=0  TranslationStandardOffsetUnits=m  TranslationROffset=0  TranslationROffsetUnits=m  TranslationThetaOffset=0  TranslationThetaOffsetUnits=deg  TranslationZOffset=0  TranslationZOffsetUnits=m
  Pose Fiche XT60 de l'ESC 4 : sm_lib/Frames and Transforms/Rigid Transform  RotationMethod=RotationMatrix  FollAlignAxisA=+X  BaseAlignAxisA=+Y  FollAlignAxisB=+Y  BaseAlignAxisB=+Z  RotationStandardAxis=+Z  RotationAngle=0  RotationAngleUnits=deg  RotationArbitraryAxis=[0 0 1]  RotationSequenceAxes=FollowerAxes  RotationSequence=XYX  RotationSequenceAngles=[0 0 0]  RotationSequenceAnglesUnits=deg  RotationMatrix=[1 0 0;0 1 0;0 0 1]  Quaternion=[1 0 0 0]  TranslationMethod=Cartesian  TranslationCartesianOffset=[-30.3 0 117.6]  TranslationCartesianOffsetUnits=mm  TranslationStandardAxis=+Z  TranslationStandardOffset=0  TranslationStandardOffsetUnits=m  TranslationROffset=0  TranslationROffsetUnits=m  TranslationThetaOffset=0  TranslationThetaOffsetUnits=deg  TranslationZOffset=0  TranslationZOffsetUnits=m
  Pose Fiche XT60 de l'alimentation : sm_lib/Frames and Transforms/Rigid Transform  RotationMethod=RotationMatrix  FollAlignAxisA=+X  BaseAlignAxisA=+Y  FollAlignAxisB=+Y  BaseAlignAxisB=+Z  RotationStandardAxis=+Z  RotationAngle=0  RotationAngleUnits=deg  RotationArbitraryAxis=[0 0 1]  RotationSequenceAxes=FollowerAxes  RotationSequence=XYX  RotationSequenceAngles=[0 0 0]  RotationSequenceAnglesUnits=deg  RotationMatrix=[0 0 1;0 -1 0;1 0 0]  Quaternion=[1 0 0 0]  TranslationMethod=Cartesian  TranslationCartesianOffset=[48.4 0 106.1]  TranslationCartesianOffsetUnits=mm  TranslationStandardAxis=+Z  TranslationStandardOffset=0  TranslationStandardOffsetUnits=m  TranslationROffset=0  TranslationROffsetUnits=m  TranslationThetaOffset=0  TranslationThetaOffsetUnits=deg  TranslationZOffset=0  TranslationZOffsetUnits=m
  Pose Tige d'équilibrage 1 : sm_lib/Frames and Transforms/Rigid Transform  RotationMethod=RotationMatrix  FollAlignAxisA=+X  BaseAlignAxisA=+Y  FollAlignAxisB=+Y  BaseAlignAxisB=+Z  RotationStandardAxis=+Z  RotationAngle=0  RotationAngleUnits=deg  RotationArbitraryAxis=[0 0 1]  RotationSequenceAxes=FollowerAxes  RotationSequence=XYX  RotationSequenceAngles=[0 0 0]  RotationSequenceAnglesUnits=deg  RotationMatrix=[0 0 1;1 0 0;0 1 0]  Quaternion=[1 0 0 0]  TranslationMethod=Cartesian  TranslationCartesianOffset=[80 25 -20]  TranslationCartesianOffsetUnits=mm  TranslationStandardAxis=+Z  TranslationStandardOffset=0  TranslationStandardOffsetUnits=m  TranslationROffset=0  TranslationROffsetUnits=m  TranslationThetaOffset=0  TranslationThetaOffsetUnits=deg  TranslationZOffset=0  TranslationZOffsetUnits=m
  Pose Tige d'équilibrage 2 : sm_lib/Frames and Transforms/Rigid Transform  RotationMethod=RotationMatrix  FollAlignAxisA=+X  BaseAlignAxisA=+Y  FollAlignAxisB=+Y  BaseAlignAxisB=+Z  RotationStandardAxis=+Z  RotationAngle=0  RotationAngleUnits=deg  RotationArbitraryAxis=[0 0 1]  RotationSequenceAxes=FollowerAxes  RotationSequence=XYX  RotationSequenceAngles=[0 0 0]  RotationSequenceAnglesUnits=deg  RotationMatrix=[-1 0 0;0 0 1;0 1 0]  Quaternion=[1 0 0 0]  TranslationMethod=Cartesian  TranslationCartesianOffset=[-25 80 -20]  TranslationCartesianOffsetUnits=mm  TranslationStandardAxis=+Z  TranslationStandardOffset=0  TranslationStandardOffsetUnits=m  TranslationROffset=0  TranslationROffsetUnits=m  TranslationThetaOffset=0  TranslationThetaOffsetUnits=deg  TranslationZOffset=0  TranslationZOffsetUnits=m
  Pose Tige d'équilibrage 3 : sm_lib/Frames and Transforms/Rigid Transform  RotationMethod=RotationMatrix  FollAlignAxisA=+X  BaseAlignAxisA=+Y  FollAlignAxisB=+Y  BaseAlignAxisB=+Z  RotationStandardAxis=+Z  RotationAngle=0  RotationAngleUnits=deg  RotationArbitraryAxis=[0 0 1]  RotationSequenceAxes=FollowerAxes  RotationSequence=XYX  RotationSequenceAngles=[0 0 0]  RotationSequenceAnglesUnits=deg  RotationMatrix=[0 0 -1;-1 0 0;0 1 0]  Quaternion=[1 0 0 0]  TranslationMethod=Cartesian  TranslationCartesianOffset=[-80 -25 -20]  TranslationCartesianOffsetUnits=mm  TranslationStandardAxis=+Z  TranslationStandardOffset=0  TranslationStandardOffsetUnits=m  TranslationROffset=0  TranslationROffsetUnits=m  TranslationThetaOffset=0  TranslationThetaOffsetUnits=deg  TranslationZOffset=0  TranslationZOffsetUnits=m
  Pose Tige d'équilibrage 4 : sm_lib/Frames and Transforms/Rigid Transform  RotationMethod=RotationMatrix  FollAlignAxisA=+X  BaseAlignAxisA=+Y  FollAlignAxisB=+Y  BaseAlignAxisB=+Z  RotationStandardAxis=+Z  RotationAngle=0  RotationAngleUnits=deg  RotationArbitraryAxis=[0 0 1]  RotationSequenceAxes=FollowerAxes  RotationSequence=XYX  RotationSequenceAngles=[0 0 0]  RotationSequenceAnglesUnits=deg  RotationMatrix=[1 0 0;0 0 -1;0 1 0]  Quaternion=[1 0 0 0]  TranslationMethod=Cartesian  TranslationCartesianOffset=[25 -80 -20]  TranslationCartesianOffsetUnits=mm  TranslationStandardAxis=+Z  TranslationStandardOffset=0  TranslationStandardOffsetUnits=m  TranslationROffset=0  TranslationROffsetUnits=m  TranslationThetaOffset=0  TranslationThetaOffsetUnits=deg  TranslationZOffset=0  TranslationZOffsetUnits=m
  Pose Écrou de réglage 1.1 : sm_lib/Frames and Transforms/Rigid Transform  RotationMethod=RotationMatrix  FollAlignAxisA=+X  BaseAlignAxisA=+Y  FollAlignAxisB=+Y  BaseAlignAxisB=+Z  RotationStandardAxis=+Z  RotationAngle=0  RotationAngleUnits=deg  RotationArbitraryAxis=[0 0 1]  RotationSequenceAxes=FollowerAxes  RotationSequence=XYX  RotationSequenceAngles=[0 0 0]  RotationSequenceAnglesUnits=deg  RotationMatrix=[0 0 1;1 0 0;0 1 0]  Quaternion=[1 0 0 0]  TranslationMethod=Cartesian  TranslationCartesianOffset=[99.9 25 -20]  TranslationCartesianOffsetUnits=mm  TranslationStandardAxis=+Z  TranslationStandardOffset=0  TranslationStandardOffsetUnits=m  TranslationROffset=0  TranslationROffsetUnits=m  TranslationThetaOffset=0  TranslationThetaOffsetUnits=deg  TranslationZOffset=0  TranslationZOffsetUnits=m
  Pose Écrou de réglage 1.2 : sm_lib/Frames and Transforms/Rigid Transform  RotationMethod=RotationMatrix  FollAlignAxisA=+X  BaseAlignAxisA=+Y  FollAlignAxisB=+Y  BaseAlignAxisB=+Z  RotationStandardAxis=+Z  RotationAngle=0  RotationAngleUnits=deg  RotationArbitraryAxis=[0 0 1]  RotationSequenceAxes=FollowerAxes  RotationSequence=XYX  RotationSequenceAngles=[0 0 0]  RotationSequenceAnglesUnits=deg  RotationMatrix=[0 0 1;1 0 0;0 1 0]  Quaternion=[1 0 0 0]  TranslationMethod=Cartesian  TranslationCartesianOffset=[104.9 25 -20]  TranslationCartesianOffsetUnits=mm  TranslationStandardAxis=+Z  TranslationStandardOffset=0  TranslationStandardOffsetUnits=m  TranslationROffset=0  TranslationROffsetUnits=m  TranslationThetaOffset=0  TranslationThetaOffsetUnits=deg  TranslationZOffset=0  TranslationZOffsetUnits=m
  Pose Écrou de réglage 1.3 : sm_lib/Frames and Transforms/Rigid Transform  RotationMethod=RotationMatrix  FollAlignAxisA=+X  BaseAlignAxisA=+Y  FollAlignAxisB=+Y  BaseAlignAxisB=+Z  RotationStandardAxis=+Z  RotationAngle=0  RotationAngleUnits=deg  RotationArbitraryAxis=[0 0 1]  RotationSequenceAxes=FollowerAxes  RotationSequence=XYX  RotationSequenceAngles=[0 0 0]  RotationSequenceAnglesUnits=deg  RotationMatrix=[0 0 1;1 0 0;0 1 0]  Quaternion=[1 0 0 0]  TranslationMethod=Cartesian  TranslationCartesianOffset=[109.9 25 -20]  TranslationCartesianOffsetUnits=mm  TranslationStandardAxis=+Z  TranslationStandardOffset=0  TranslationStandardOffsetUnits=m  TranslationROffset=0  TranslationROffsetUnits=m  TranslationThetaOffset=0  TranslationThetaOffsetUnits=deg  TranslationZOffset=0  TranslationZOffsetUnits=m
  Pose Écrou de réglage 2.1 : sm_lib/Frames and Transforms/Rigid Transform  RotationMethod=RotationMatrix  FollAlignAxisA=+X  BaseAlignAxisA=+Y  FollAlignAxisB=+Y  BaseAlignAxisB=+Z  RotationStandardAxis=+Z  RotationAngle=0  RotationAngleUnits=deg  RotationArbitraryAxis=[0 0 1]  RotationSequenceAxes=FollowerAxes  RotationSequence=XYX  RotationSequenceAngles=[0 0 0]  RotationSequenceAnglesUnits=deg  RotationMatrix=[-1 0 0;0 0 1;0 1 0]  Quaternion=[1 0 0 0]  TranslationMethod=Cartesian  TranslationCartesianOffset=[-25 89.1 -20]  TranslationCartesianOffsetUnits=mm  TranslationStandardAxis=+Z  TranslationStandardOffset=0  TranslationStandardOffsetUnits=m  TranslationROffset=0  TranslationROffsetUnits=m  TranslationThetaOffset=0  TranslationThetaOffsetUnits=deg  TranslationZOffset=0  TranslationZOffsetUnits=m
  Pose Écrou de réglage 4.1 : sm_lib/Frames and Transforms/Rigid Transform  RotationMethod=RotationMatrix  FollAlignAxisA=+X  BaseAlignAxisA=+Y  FollAlignAxisB=+Y  BaseAlignAxisB=+Z  RotationStandardAxis=+Z  RotationAngle=0  RotationAngleUnits=deg  RotationArbitraryAxis=[0 0 1]  RotationSequenceAxes=FollowerAxes  RotationSequence=XYX  RotationSequenceAngles=[0 0 0]  RotationSequenceAnglesUnits=deg  RotationMatrix=[1 0 0;0 0 -1;0 1 0]  Quaternion=[1 0 0 0]  TranslationMethod=Cartesian  TranslationCartesianOffset=[25 -101.1 -20]  TranslationCartesianOffsetUnits=mm  TranslationStandardAxis=+Z  TranslationStandardOffset=0  TranslationStandardOffsetUnits=m  TranslationROffset=0  TranslationROffsetUnits=m  TranslationThetaOffset=0  TranslationThetaOffsetUnits=deg  TranslationZOffset=0  TranslationZOffsetUnits=m
  Pose Écrou de réglage 4.2 : sm_lib/Frames and Transforms/Rigid Transform  RotationMethod=RotationMatrix  FollAlignAxisA=+X  BaseAlignAxisA=+Y  FollAlignAxisB=+Y  BaseAlignAxisB=+Z  RotationStandardAxis=+Z  RotationAngle=0  RotationAngleUnits=deg  RotationArbitraryAxis=[0 0 1]  RotationSequenceAxes=FollowerAxes  RotationSequence=XYX  RotationSequenceAngles=[0 0 0]  RotationSequenceAnglesUnits=deg  RotationMatrix=[1 0 0;0 0 -1;0 1 0]  Quaternion=[1 0 0 0]  TranslationMethod=Cartesian  TranslationCartesianOffset=[25 -106.1 -20]  TranslationCartesianOffsetUnits=mm  TranslationStandardAxis=+Z  TranslationStandardOffset=0  TranslationStandardOffsetUnits=m  TranslationROffset=0  TranslationROffsetUnits=m  TranslationThetaOffset=0  TranslationThetaOffsetUnits=deg  TranslationZOffset=0  TranslationZOffsetUnits=m
  Pose Écrou de serrage extérieur 1 : sm_lib/Frames and Transforms/Rigid Transform  RotationMethod=RotationMatrix  FollAlignAxisA=+X  BaseAlignAxisA=+Y  FollAlignAxisB=+Y  BaseAlignAxisB=+Z  RotationStandardAxis=+Z  RotationAngle=0  RotationAngleUnits=deg  RotationArbitraryAxis=[0 0 1]  RotationSequenceAxes=FollowerAxes  RotationSequence=XYX  RotationSequenceAngles=[0 0 0]  RotationSequenceAnglesUnits=deg  RotationMatrix=[0 0 1;1 0 0;0 1 0]  Quaternion=[1 0 0 0]  TranslationMethod=Cartesian  TranslationCartesianOffset=[82.5 25 -20]  TranslationCartesianOffsetUnits=mm  TranslationStandardAxis=+Z  TranslationStandardOffset=0  TranslationStandardOffsetUnits=m  TranslationROffset=0  TranslationROffsetUnits=m  TranslationThetaOffset=0  TranslationThetaOffsetUnits=deg  TranslationZOffset=0  TranslationZOffsetUnits=m
  Pose Écrou de serrage extérieur 2 : sm_lib/Frames and Transforms/Rigid Transform  RotationMethod=RotationMatrix  FollAlignAxisA=+X  BaseAlignAxisA=+Y  FollAlignAxisB=+Y  BaseAlignAxisB=+Z  RotationStandardAxis=+Z  RotationAngle=0  RotationAngleUnits=deg  RotationArbitraryAxis=[0 0 1]  RotationSequenceAxes=FollowerAxes  RotationSequence=XYX  RotationSequenceAngles=[0 0 0]  RotationSequenceAnglesUnits=deg  RotationMatrix=[-1 0 0;0 0 1;0 1 0]  Quaternion=[1 0 0 0]  TranslationMethod=Cartesian  TranslationCartesianOffset=[-25 82.5 -20]  TranslationCartesianOffsetUnits=mm  TranslationStandardAxis=+Z  TranslationStandardOffset=0  TranslationStandardOffsetUnits=m  TranslationROffset=0  TranslationROffsetUnits=m  TranslationThetaOffset=0  TranslationThetaOffsetUnits=deg  TranslationZOffset=0  TranslationZOffsetUnits=m
  Pose Écrou de serrage extérieur 3 : sm_lib/Frames and Transforms/Rigid Transform  RotationMethod=RotationMatrix  FollAlignAxisA=+X  BaseAlignAxisA=+Y  FollAlignAxisB=+Y  BaseAlignAxisB=+Z  RotationStandardAxis=+Z  RotationAngle=0  RotationAngleUnits=deg  RotationArbitraryAxis=[0 0 1]  RotationSequenceAxes=FollowerAxes  RotationSequence=XYX  RotationSequenceAngles=[0 0 0]  RotationSequenceAnglesUnits=deg  RotationMatrix=[0 0 -1;-1 0 0;0 1 0]  Quaternion=[1 0 0 0]  TranslationMethod=Cartesian  TranslationCartesianOffset=[-82.5 -25 -20]  TranslationCartesianOffsetUnits=mm  TranslationStandardAxis=+Z  TranslationStandardOffset=0  TranslationStandardOffsetUnits=m  TranslationROffset=0  TranslationROffsetUnits=m  TranslationThetaOffset=0  TranslationThetaOffsetUnits=deg  TranslationZOffset=0  TranslationZOffsetUnits=m
  Pose Écrou de serrage extérieur 4 : sm_lib/Frames and Transforms/Rigid Transform  RotationMethod=RotationMatrix  FollAlignAxisA=+X  BaseAlignAxisA=+Y  FollAlignAxisB=+Y  BaseAlignAxisB=+Z  RotationStandardAxis=+Z  RotationAngle=0  RotationAngleUnits=deg  RotationArbitraryAxis=[0 0 1]  RotationSequenceAxes=FollowerAxes  RotationSequence=XYX  RotationSequenceAngles=[0 0 0]  RotationSequenceAnglesUnits=deg  RotationMatrix=[1 0 0;0 0 -1;0 1 0]  Quaternion=[1 0 0 0]  TranslationMethod=Cartesian  TranslationCartesianOffset=[25 -82.5 -20]  TranslationCartesianOffsetUnits=mm  TranslationStandardAxis=+Z  TranslationStandardOffset=0  TranslationStandardOffsetUnits=m  TranslationROffset=0  TranslationROffsetUnits=m  TranslationThetaOffset=0  TranslationThetaOffsetUnits=deg  TranslationZOffset=0  TranslationZOffsetUnits=m
  Pose Écrou de serrage intérieur 1 : sm_lib/Frames and Transforms/Rigid Transform  RotationMethod=RotationMatrix  FollAlignAxisA=+X  BaseAlignAxisA=+Y  FollAlignAxisB=+Y  BaseAlignAxisB=+Z  RotationStandardAxis=+Z  RotationAngle=0  RotationAngleUnits=deg  RotationArbitraryAxis=[0 0 1]  RotationSequenceAxes=FollowerAxes  RotationSequence=XYX  RotationSequenceAngles=[0 0 0]  RotationSequenceAnglesUnits=deg  RotationMatrix=[0 0 1;1 0 0;0 1 0]  Quaternion=[1 0 0 0]  TranslationMethod=Cartesian  TranslationCartesianOffset=[73.5 25 -20]  TranslationCartesianOffsetUnits=mm  TranslationStandardAxis=+Z  TranslationStandardOffset=0  TranslationStandardOffsetUnits=m  TranslationROffset=0  TranslationROffsetUnits=m  TranslationThetaOffset=0  TranslationThetaOffsetUnits=deg  TranslationZOffset=0  TranslationZOffsetUnits=m
  Pose Écrou de serrage intérieur 2 : sm_lib/Frames and Transforms/Rigid Transform  RotationMethod=RotationMatrix  FollAlignAxisA=+X  BaseAlignAxisA=+Y  FollAlignAxisB=+Y  BaseAlignAxisB=+Z  RotationStandardAxis=+Z  RotationAngle=0  RotationAngleUnits=deg  RotationArbitraryAxis=[0 0 1]  RotationSequenceAxes=FollowerAxes  RotationSequence=XYX  RotationSequenceAngles=[0 0 0]  RotationSequenceAnglesUnits=deg  RotationMatrix=[-1 0 0;0 0 1;0 1 0]  Quaternion=[1 0 0 0]  TranslationMethod=Cartesian  TranslationCartesianOffset=[-25 73.5 -20]  TranslationCartesianOffsetUnits=mm  TranslationStandardAxis=+Z  TranslationStandardOffset=0  TranslationStandardOffsetUnits=m  TranslationROffset=0  TranslationROffsetUnits=m  TranslationThetaOffset=0  TranslationThetaOffsetUnits=deg  TranslationZOffset=0  TranslationZOffsetUnits=m
  Pose Écrou de serrage intérieur 3 : sm_lib/Frames and Transforms/Rigid Transform  RotationMethod=RotationMatrix  FollAlignAxisA=+X  BaseAlignAxisA=+Y  FollAlignAxisB=+Y  BaseAlignAxisB=+Z  RotationStandardAxis=+Z  RotationAngle=0  RotationAngleUnits=deg  RotationArbitraryAxis=[0 0 1]  RotationSequenceAxes=FollowerAxes  RotationSequence=XYX  RotationSequenceAngles=[0 0 0]  RotationSequenceAnglesUnits=deg  RotationMatrix=[0 0 -1;-1 0 0;0 1 0]  Quaternion=[1 0 0 0]  TranslationMethod=Cartesian  TranslationCartesianOffset=[-73.5 -25 -20]  TranslationCartesianOffsetUnits=mm  TranslationStandardAxis=+Z  TranslationStandardOffset=0  TranslationStandardOffsetUnits=m  TranslationROffset=0  TranslationROffsetUnits=m  TranslationThetaOffset=0  TranslationThetaOffsetUnits=deg  TranslationZOffset=0  TranslationZOffsetUnits=m
  Pose Écrou de serrage intérieur 4 : sm_lib/Frames and Transforms/Rigid Transform  RotationMethod=RotationMatrix  FollAlignAxisA=+X  BaseAlignAxisA=+Y  FollAlignAxisB=+Y  BaseAlignAxisB=+Z  RotationStandardAxis=+Z  RotationAngle=0  RotationAngleUnits=deg  RotationArbitraryAxis=[0 0 1]  RotationSequenceAxes=FollowerAxes  RotationSequence=XYX  RotationSequenceAngles=[0 0 0]  RotationSequenceAnglesUnits=deg  RotationMatrix=[1 0 0;0 0 -1;0 1 0]  Quaternion=[1 0 0 0]  TranslationMethod=Cartesian  TranslationCartesianOffset=[25 -73.5 -20]  TranslationCartesianOffsetUnits=mm  TranslationStandardAxis=+Z  TranslationStandardOffset=0  TranslationStandardOffsetUnits=m  TranslationROffset=0  TranslationROffsetUnits=m  TranslationThetaOffset=0  TranslationThetaOffsetUnits=deg  TranslationZOffset=0  TranslationZOffsetUnits=m
  RW-50_Fils-moteur : sm_lib/Body Elements/File Solid  Description=|  ExtGeomFileName=RW-50_Fils-moteur.stl  UnitType=Custom  ExtGeomFileUnits=mm  StepReaderType=HEX  ExportConvexHullGeometry=off  InertiaType=Custom  BasedOnType=DensityFromFile  Density=1000  DensityUnits=kg/m^3  Mass=0.03888  MassUnits=kg  CenterOfMass=[-2.3601672e-18 -2.1013102e-17 0.020821505]  CenterOfMassUnits=m  MomentsOfInertia=[0.0001300214 0.0001300214 0.0001919552]  MomentsOfInertiaUnits=kg*m^2  ProductsOfInertia=[-9.054182e-21 1.2297861e-20 -2.500698e-20]  ProductsOfInertiaUnits=kg*m^2  GraphicType=FromGeometry  MarkerShape=Sphere  MarkerSize=10  GraphicVisPropType=SimpleVisualProperties  GraphicDiffuseColor=[0.18 0.373 0.816]  GraphicOpacity=1  GraphicSpecularColor=[0.5 0.5 0.5 1.0]  GraphicAmbientColor=[0.15 0.15 0.15 1.0]  GraphicEmissiveColor=[0.0 0.0 0.0 1.0]  GraphicShininess=75  DoExposeReferenceFrame=on  SerializedFrames=<Frames/>
      | Pièce CAO : RW-50_Fils-moteur (RW-50_Fils-moteur)
      | Masse 38.88 g : 4 faisceaux de 3 fils 16 AWG silicone de 180 mm, 54 g/m.
      | Centre de masse et inertie : calculés sur la géométrie de la CAO.
  RW-51_Fils-alim-ESC : sm_lib/Body Elements/File Solid  Description=|  ExtGeomFileName=RW-51_Fils-alim-ESC.stl  UnitType=Custom  ExtGeomFileUnits=mm  StepReaderType=HEX  ExportConvexHullGeometry=off  InertiaType=Custom  BasedOnType=DensityFromFile  Density=1000  DensityUnits=kg/m^3  Mass=0.01872  MassUnits=kg  CenterOfMass=[-0.0033865484 -5.9308914e-05 0.12828728]  CenterOfMassUnits=m  MomentsOfInertia=[2.7716326e-05 3.3143726e-05 4.3554182e-05]  MomentsOfInertiaUnits=kg*m^2  ProductsOfInertia=[-4.3478411e-08 1.3746238e-06 -8.4492914e-07]  ProductsOfInertiaUnits=kg*m^2  GraphicType=FromGeometry  MarkerShape=Sphere  MarkerSize=10  GraphicVisPropType=SimpleVisualProperties  GraphicDiffuseColor=[0.816 0.188 0.188]  GraphicOpacity=1  GraphicSpecularColor=[0.5 0.5 0.5 1.0]  GraphicAmbientColor=[0.15 0.15 0.15 1.0]  GraphicEmissiveColor=[0.0 0.0 0.0 1.0]  GraphicShininess=75  DoExposeReferenceFrame=on  SerializedFrames=<Frames/>
      | Pièce CAO : RW-51_Fils-alim-ESC (RW-51_Fils-alim-ESC)
      | Masse 18.72 g : 4 paires de fils 16 AWG silicone de 130 mm, 36 g/m.
      | Centre de masse et inertie : calculés sur la géométrie de la CAO.
  RW-52_Cable-alimentation : sm_lib/Body Elements/File Solid  Description=|  ExtGeomFileName=RW-52_Cable-alimentation.stl  UnitType=Custom  ExtGeomFileUnits=mm  StepReaderType=HEX  ExportConvexHullGeometry=off  InertiaType=Custom  BasedOnType=DensityFromFile  Density=1000  DensityUnits=kg/m^3  Mass=0.0056208194  MassUnits=kg  CenterOfMass=[0.08398819 -0.014370123 0.043424373]  CenterOfMassUnits=m  MomentsOfInertia=[1.076798e-05 1.0543406e-05 4.5472331e-07]  MomentsOfInertiaUnits=kg*m^2  ProductsOfInertia=[-1.7525173e-06 4.2510825e-07 1.0764224e-07]  ProductsOfInertiaUnits=kg*m^2  GraphicType=FromGeometry  MarkerShape=Sphere  MarkerSize=10  GraphicVisPropType=SimpleVisualProperties  GraphicDiffuseColor=[0.627 0.125 0.125]  GraphicOpacity=1  GraphicSpecularColor=[0.5 0.5 0.5 1.0]  GraphicAmbientColor=[0.15 0.15 0.15 1.0]  GraphicEmissiveColor=[0.0 0.0 0.0 1.0]  GraphicShininess=75  DoExposeReferenceFrame=on  SerializedFrames=<Frames/>
      | Pièce CAO : RW-52_Cable-alimentation (RW-52_Cable-alimentation)
      | Masse 5.62 g : câble d'alimentation, 2 fils 16 AWG, partie portée par le dispositif, 36 g/m.
      | Centre de masse et inertie : calculés sur la géométrie de la CAO.
  RW-53_Cables-commande-ESC : sm_lib/Body Elements/File Solid  Description=|  ExtGeomFileName=RW-53_Cables-commande-ESC.stl  UnitType=Custom  ExtGeomFileUnits=mm  StepReaderType=HEX  ExportConvexHullGeometry=off  InertiaType=Custom  BasedOnType=DensityFromFile  Density=1000  DensityUnits=kg/m^3  Mass=0.0066822094  MassUnits=kg  CenterOfMass=[-0.038949445 -0.0015750344 0.082767272]  CenterOfMassUnits=m  MomentsOfInertia=[2.0593621e-05 1.4501798e-05 3.224252e-05]  MomentsOfInertiaUnits=kg*m^2  ProductsOfInertia=[-8.6494731e-08 2.9330664e-06 4.3469975e-07]  ProductsOfInertiaUnits=kg*m^2  GraphicType=FromGeometry  MarkerShape=Sphere  MarkerSize=10  GraphicVisPropType=SimpleVisualProperties  GraphicDiffuseColor=[0.89 0.467 0.761]  GraphicOpacity=1  GraphicSpecularColor=[0.5 0.5 0.5 1.0]  GraphicAmbientColor=[0.15 0.15 0.15 1.0]  GraphicEmissiveColor=[0.0 0.0 0.0 1.0]  GraphicShininess=75  DoExposeReferenceFrame=on  SerializedFrames=<Frames/>
      | Pièce CAO : RW-53_Cables-commande-ESC (RW-53_Cables-commande-ESC)
      | Masse 6.68 g : 4 câbles de commande à 3 fils, 10 g/m.
      | Centre de masse et inertie : calculés sur la géométrie de la CAO.
  RW-54_Cables-capteurs : sm_lib/Body Elements/File Solid  Description=|  ExtGeomFileName=RW-54_Cables-capteurs.stl  UnitType=Custom  ExtGeomFileUnits=mm  StepReaderType=HEX  ExportConvexHullGeometry=off  InertiaType=Custom  BasedOnType=DensityFromFile  Density=1000  DensityUnits=kg/m^3  Mass=0.009767313  MassUnits=kg  CenterOfMass=[-0.024243272 0.00271566 0.07359388]  CenterOfMassUnits=m  MomentsOfInertia=[4.8602722e-05 4.7850178e-05 9.2264301e-05]  MomentsOfInertiaUnits=kg*m^2  ProductsOfInertia=[6.7933339e-08 3.8144014e-06 -7.0003929e-07]  ProductsOfInertiaUnits=kg*m^2  GraphicType=FromGeometry  MarkerShape=Sphere  MarkerSize=10  GraphicVisPropType=SimpleVisualProperties  GraphicDiffuseColor=[0.09 0.745 0.812]  GraphicOpacity=1  GraphicSpecularColor=[0.5 0.5 0.5 1.0]  GraphicAmbientColor=[0.15 0.15 0.15 1.0]  GraphicEmissiveColor=[0.0 0.0 0.0 1.0]  GraphicShininess=75  DoExposeReferenceFrame=on  SerializedFrames=<Frames/>
      | Pièce CAO : RW-54_Cables-capteurs (RW-54_Cables-capteurs)
      | Masse 9.77 g : 4 câbles de capteur à 3 fils Dupont, 9 g/m.
      | Centre de masse et inertie : calculés sur la géométrie de la CAO.
  RW-55_Cable-BNO055 : sm_lib/Body Elements/File Solid  Description=|  ExtGeomFileName=RW-55_Cable-BNO055.stl  UnitType=Custom  ExtGeomFileUnits=mm  StepReaderType=HEX  ExportConvexHullGeometry=off  InertiaType=Custom  BasedOnType=DensityFromFile  Density=1000  DensityUnits=kg/m^3  Mass=0.0028855989  MassUnits=kg  CenterOfMass=[-0.07536581 0.0023570075 0.059637144]  CenterOfMassUnits=m  MomentsOfInertia=[5.203349e-06 7.2534899e-06 2.1252872e-06]  MomentsOfInertiaUnits=kg*m^2  ProductsOfInertia=[3.8915225e-07 -1.1533421e-06 6.0461993e-08]  ProductsOfInertiaUnits=kg*m^2  GraphicType=FromGeometry  MarkerShape=Sphere  MarkerSize=10  GraphicVisPropType=SimpleVisualProperties  GraphicDiffuseColor=[0.173 0.627 0.173]  GraphicOpacity=1  GraphicSpecularColor=[0.5 0.5 0.5 1.0]  GraphicAmbientColor=[0.15 0.15 0.15 1.0]  GraphicEmissiveColor=[0.0 0.0 0.0 1.0]  GraphicShininess=75  DoExposeReferenceFrame=on  SerializedFrames=<Frames/>
      | Pièce CAO : RW-55_Cable-BNO055 (RW-55_Cable-BNO055)
      | Masse 2.89 g : 4 fils Dupont du BNO055, partie portée par le dispositif, 12 g/m.
      | Centre de masse et inertie : calculés sur la géométrie de la CAO.
  RW-56_Nappe-signaux : sm_lib/Body Elements/File Solid  Description=|  ExtGeomFileName=RW-56_Nappe-signaux.stl  UnitType=Custom  ExtGeomFileUnits=mm  StepReaderType=HEX  ExportConvexHullGeometry=off  InertiaType=Custom  BasedOnType=DensityFromFile  Density=1000  DensityUnits=kg/m^3  Mass=0.004085389  MassUnits=kg  CenterOfMass=[-0.086476462 0.018940386 0.010903026]  CenterOfMassUnits=m  MomentsOfInertia=[2.5472691e-06 2.4116489e-06 1.7814745e-07]  MomentsOfInertiaUnits=kg*m^2  ProductsOfInertia=[3.8568249e-07 9.8062325e-08 -1.8987217e-08]  ProductsOfInertiaUnits=kg*m^2  GraphicType=FromGeometry  MarkerShape=Sphere  MarkerSize=10  GraphicVisPropType=SimpleVisualProperties  GraphicDiffuseColor=[0.58 0.404 0.741]  GraphicOpacity=1  GraphicSpecularColor=[0.5 0.5 0.5 1.0]  GraphicAmbientColor=[0.15 0.15 0.15 1.0]  GraphicEmissiveColor=[0.0 0.0 0.0 1.0]  GraphicShininess=75  DoExposeReferenceFrame=on  SerializedFrames=<Frames/>
      | Pièce CAO : RW-56_Nappe-signaux (RW-56_Nappe-signaux)
      | Masse 4.09 g : nappe des signaux, partie portée par le dispositif, 45 g/m.
      | Centre de masse et inertie : calculés sur la géométrie de la CAO.
  Tige d'équilibrage 1 : sm_lib/Body Elements/File Solid  Description=|  ExtGeomFileName=RW-40_Tige-filetee-M6x60.stl  UnitType=Custom  ExtGeomFileUnits=mm  StepReaderType=HEX  ExportConvexHullGeometry=off  InertiaType=Custom  BasedOnType=DensityFromFile  Density=1000  DensityUnits=kg/m^3  Mass=0.0106  MassUnits=kg  CenterOfMass=[-1.1727477e-19 1.0875012e-19 0.0195]  CenterOfMassUnits=m  MomentsOfInertia=[3.20385e-06 3.20385e-06 4.77e-08]  MomentsOfInertiaUnits=kg*m^2  ProductsOfInertia=[3.26899e-25 -7.1922943e-24 2.9502635e-25]  ProductsOfInertiaUnits=kg*m^2  GraphicType=FromGeometry  MarkerShape=Sphere  MarkerSize=10  GraphicVisPropType=SimpleVisualProperties  GraphicDiffuseColor=[0.604 0.604 0.604]  GraphicOpacity=1  GraphicSpecularColor=[0.5 0.5 0.5 1.0]  GraphicAmbientColor=[0.15 0.15 0.15 1.0]  GraphicEmissiveColor=[0.0 0.0 0.0 1.0]  GraphicShininess=75  DoExposeReferenceFrame=on  SerializedFrames=<Frames/>
      | Pièce CAO : Tige d'équilibrage 1 (RW-40_Tige-filetee-M6x60)
      | Masse 10.60 g : tige filetée M6 × 60 en acier, 10,6 g (0,177 g/mm).
      | Centre de masse et inertie : calculés sur la géométrie de la CAO.
  Tige d'équilibrage 2 : sm_lib/Body Elements/File Solid  Description=|  ExtGeomFileName=RW-40_Tige-filetee-M6x60.stl  UnitType=Custom  ExtGeomFileUnits=mm  StepReaderType=HEX  ExportConvexHullGeometry=off  InertiaType=Custom  BasedOnType=DensityFromFile  Density=1000  DensityUnits=kg/m^3  Mass=0.0106  MassUnits=kg  CenterOfMass=[-1.1727477e-19 1.0875012e-19 0.0195]  CenterOfMassUnits=m  MomentsOfInertia=[3.20385e-06 3.20385e-06 4.77e-08]  MomentsOfInertiaUnits=kg*m^2  ProductsOfInertia=[3.26899e-25 -7.1922943e-24 2.9502635e-25]  ProductsOfInertiaUnits=kg*m^2  GraphicType=FromGeometry  MarkerShape=Sphere  MarkerSize=10  GraphicVisPropType=SimpleVisualProperties  GraphicDiffuseColor=[0.604 0.604 0.604]  GraphicOpacity=1  GraphicSpecularColor=[0.5 0.5 0.5 1.0]  GraphicAmbientColor=[0.15 0.15 0.15 1.0]  GraphicEmissiveColor=[0.0 0.0 0.0 1.0]  GraphicShininess=75  DoExposeReferenceFrame=on  SerializedFrames=<Frames/>
      | Pièce CAO : Tige d'équilibrage 2 (RW-40_Tige-filetee-M6x60)
      | Masse 10.60 g : tige filetée M6 × 60 en acier, 10,6 g (0,177 g/mm).
      | Centre de masse et inertie : calculés sur la géométrie de la CAO.
  Tige d'équilibrage 3 : sm_lib/Body Elements/File Solid  Description=|  ExtGeomFileName=RW-40_Tige-filetee-M6x60.stl  UnitType=Custom  ExtGeomFileUnits=mm  StepReaderType=HEX  ExportConvexHullGeometry=off  InertiaType=Custom  BasedOnType=DensityFromFile  Density=1000  DensityUnits=kg/m^3  Mass=0.0106  MassUnits=kg  CenterOfMass=[-1.1727477e-19 1.0875012e-19 0.0195]  CenterOfMassUnits=m  MomentsOfInertia=[3.20385e-06 3.20385e-06 4.77e-08]  MomentsOfInertiaUnits=kg*m^2  ProductsOfInertia=[3.26899e-25 -7.1922943e-24 2.9502635e-25]  ProductsOfInertiaUnits=kg*m^2  GraphicType=FromGeometry  MarkerShape=Sphere  MarkerSize=10  GraphicVisPropType=SimpleVisualProperties  GraphicDiffuseColor=[0.604 0.604 0.604]  GraphicOpacity=1  GraphicSpecularColor=[0.5 0.5 0.5 1.0]  GraphicAmbientColor=[0.15 0.15 0.15 1.0]  GraphicEmissiveColor=[0.0 0.0 0.0 1.0]  GraphicShininess=75  DoExposeReferenceFrame=on  SerializedFrames=<Frames/>
      | Pièce CAO : Tige d'équilibrage 3 (RW-40_Tige-filetee-M6x60)
      | Masse 10.60 g : tige filetée M6 × 60 en acier, 10,6 g (0,177 g/mm).
      | Centre de masse et inertie : calculés sur la géométrie de la CAO.
  Tige d'équilibrage 4 : sm_lib/Body Elements/File Solid  Description=|  ExtGeomFileName=RW-40_Tige-filetee-M6x60.stl  UnitType=Custom  ExtGeomFileUnits=mm  StepReaderType=HEX  ExportConvexHullGeometry=off  InertiaType=Custom  BasedOnType=DensityFromFile  Density=1000  DensityUnits=kg/m^3  Mass=0.0106  MassUnits=kg  CenterOfMass=[-1.1727477e-19 1.0875012e-19 0.0195]  CenterOfMassUnits=m  MomentsOfInertia=[3.20385e-06 3.20385e-06 4.77e-08]  MomentsOfInertiaUnits=kg*m^2  ProductsOfInertia=[3.26899e-25 -7.1922943e-24 2.9502635e-25]  ProductsOfInertiaUnits=kg*m^2  GraphicType=FromGeometry  MarkerShape=Sphere  MarkerSize=10  GraphicVisPropType=SimpleVisualProperties  GraphicDiffuseColor=[0.604 0.604 0.604]  GraphicOpacity=1  GraphicSpecularColor=[0.5 0.5 0.5 1.0]  GraphicAmbientColor=[0.15 0.15 0.15 1.0]  GraphicEmissiveColor=[0.0 0.0 0.0 1.0]  GraphicShininess=75  DoExposeReferenceFrame=on  SerializedFrames=<Frames/>
      | Pièce CAO : Tige d'équilibrage 4 (RW-40_Tige-filetee-M6x60)
      | Masse 10.60 g : tige filetée M6 × 60 en acier, 10,6 g (0,177 g/mm).
      | Centre de masse et inertie : calculés sur la géométrie de la CAO.
  Écrou de réglage 1.1 : sm_lib/Body Elements/File Solid  Description=|  ExtGeomFileName=RW-41_Ecrou-M6.stl  UnitType=Custom  ExtGeomFileUnits=mm  StepReaderType=HEX  ExportConvexHullGeometry=off  InertiaType=Custom  BasedOnType=DensityFromFile  Density=1000  DensityUnits=kg/m^3  Mass=0.0024  MassUnits=kg  CenterOfMass=[1.6445434e-19 4.9031279e-19 -1.3524518e-36]  CenterOfMassUnits=m  MomentsOfInertia=[2.7128132e-08 2.7128132e-08 4.4256265e-08]  MomentsOfInertiaUnits=kg*m^2  ProductsOfInertia=[-1.5470275e-25 1.3498961e-25 -3.9289691e-24]  ProductsOfInertiaUnits=kg*m^2  GraphicType=FromGeometry  MarkerShape=Sphere  MarkerSize=10  GraphicVisPropType=SimpleVisualProperties  GraphicDiffuseColor=[0.788 0.635 0.153]  GraphicOpacity=1  GraphicSpecularColor=[0.5 0.5 0.5 1.0]  GraphicAmbientColor=[0.15 0.15 0.15 1.0]  GraphicEmissiveColor=[0.0 0.0 0.0 1.0]  GraphicShininess=75  DoExposeReferenceFrame=on  SerializedFrames=<Frames/>
      | Pièce CAO : Écrou de réglage 1.1 (RW-41_Ecrou-M6)
      | Masse 2.40 g : écrou hexagonal M6 en acier, 2,4 g.
      | Centre de masse et inertie : calculés sur la géométrie de la CAO.
  Écrou de réglage 1.2 : sm_lib/Body Elements/File Solid  Description=|  ExtGeomFileName=RW-41_Ecrou-M6.stl  UnitType=Custom  ExtGeomFileUnits=mm  StepReaderType=HEX  ExportConvexHullGeometry=off  InertiaType=Custom  BasedOnType=DensityFromFile  Density=1000  DensityUnits=kg/m^3  Mass=0.0024  MassUnits=kg  CenterOfMass=[1.6445434e-19 4.9031279e-19 -1.3524518e-36]  CenterOfMassUnits=m  MomentsOfInertia=[2.7128132e-08 2.7128132e-08 4.4256265e-08]  MomentsOfInertiaUnits=kg*m^2  ProductsOfInertia=[-1.5470275e-25 1.3498961e-25 -3.9289691e-24]  ProductsOfInertiaUnits=kg*m^2  GraphicType=FromGeometry  MarkerShape=Sphere  MarkerSize=10  GraphicVisPropType=SimpleVisualProperties  GraphicDiffuseColor=[0.788 0.635 0.153]  GraphicOpacity=1  GraphicSpecularColor=[0.5 0.5 0.5 1.0]  GraphicAmbientColor=[0.15 0.15 0.15 1.0]  GraphicEmissiveColor=[0.0 0.0 0.0 1.0]  GraphicShininess=75  DoExposeReferenceFrame=on  SerializedFrames=<Frames/>
      | Pièce CAO : Écrou de réglage 1.2 (RW-41_Ecrou-M6)
      | Masse 2.40 g : écrou hexagonal M6 en acier, 2,4 g.
      | Centre de masse et inertie : calculés sur la géométrie de la CAO.
  Écrou de réglage 1.3 : sm_lib/Body Elements/File Solid  Description=|  ExtGeomFileName=RW-41_Ecrou-M6.stl  UnitType=Custom  ExtGeomFileUnits=mm  StepReaderType=HEX  ExportConvexHullGeometry=off  InertiaType=Custom  BasedOnType=DensityFromFile  Density=1000  DensityUnits=kg/m^3  Mass=0.0024  MassUnits=kg  CenterOfMass=[1.6445434e-19 4.9031279e-19 -1.3524518e-36]  CenterOfMassUnits=m  MomentsOfInertia=[2.7128132e-08 2.7128132e-08 4.4256265e-08]  MomentsOfInertiaUnits=kg*m^2  ProductsOfInertia=[-1.5470275e-25 1.3498961e-25 -3.9289691e-24]  ProductsOfInertiaUnits=kg*m^2  GraphicType=FromGeometry  MarkerShape=Sphere  MarkerSize=10  GraphicVisPropType=SimpleVisualProperties  GraphicDiffuseColor=[0.788 0.635 0.153]  GraphicOpacity=1  GraphicSpecularColor=[0.5 0.5 0.5 1.0]  GraphicAmbientColor=[0.15 0.15 0.15 1.0]  GraphicEmissiveColor=[0.0 0.0 0.0 1.0]  GraphicShininess=75  DoExposeReferenceFrame=on  SerializedFrames=<Frames/>
      | Pièce CAO : Écrou de réglage 1.3 (RW-41_Ecrou-M6)
      | Masse 2.40 g : écrou hexagonal M6 en acier, 2,4 g.
      | Centre de masse et inertie : calculés sur la géométrie de la CAO.
  Écrou de réglage 2.1 : sm_lib/Body Elements/File Solid  Description=|  ExtGeomFileName=RW-41_Ecrou-M6.stl  UnitType=Custom  ExtGeomFileUnits=mm  StepReaderType=HEX  ExportConvexHullGeometry=off  InertiaType=Custom  BasedOnType=DensityFromFile  Density=1000  DensityUnits=kg/m^3  Mass=0.0024  MassUnits=kg  CenterOfMass=[1.6445434e-19 4.9031279e-19 -1.3524518e-36]  CenterOfMassUnits=m  MomentsOfInertia=[2.7128132e-08 2.7128132e-08 4.4256265e-08]  MomentsOfInertiaUnits=kg*m^2  ProductsOfInertia=[-1.5470275e-25 1.3498961e-25 -3.9289691e-24]  ProductsOfInertiaUnits=kg*m^2  GraphicType=FromGeometry  MarkerShape=Sphere  MarkerSize=10  GraphicVisPropType=SimpleVisualProperties  GraphicDiffuseColor=[0.788 0.635 0.153]  GraphicOpacity=1  GraphicSpecularColor=[0.5 0.5 0.5 1.0]  GraphicAmbientColor=[0.15 0.15 0.15 1.0]  GraphicEmissiveColor=[0.0 0.0 0.0 1.0]  GraphicShininess=75  DoExposeReferenceFrame=on  SerializedFrames=<Frames/>
      | Pièce CAO : Écrou de réglage 2.1 (RW-41_Ecrou-M6)
      | Masse 2.40 g : écrou hexagonal M6 en acier, 2,4 g.
      | Centre de masse et inertie : calculés sur la géométrie de la CAO.
  Écrou de réglage 4.1 : sm_lib/Body Elements/File Solid  Description=|  ExtGeomFileName=RW-41_Ecrou-M6.stl  UnitType=Custom  ExtGeomFileUnits=mm  StepReaderType=HEX  ExportConvexHullGeometry=off  InertiaType=Custom  BasedOnType=DensityFromFile  Density=1000  DensityUnits=kg/m^3  Mass=0.0024  MassUnits=kg  CenterOfMass=[1.6445434e-19 4.9031279e-19 -1.3524518e-36]  CenterOfMassUnits=m  MomentsOfInertia=[2.7128132e-08 2.7128132e-08 4.4256265e-08]  MomentsOfInertiaUnits=kg*m^2  ProductsOfInertia=[-1.5470275e-25 1.3498961e-25 -3.9289691e-24]  ProductsOfInertiaUnits=kg*m^2  GraphicType=FromGeometry  MarkerShape=Sphere  MarkerSize=10  GraphicVisPropType=SimpleVisualProperties  GraphicDiffuseColor=[0.788 0.635 0.153]  GraphicOpacity=1  GraphicSpecularColor=[0.5 0.5 0.5 1.0]  GraphicAmbientColor=[0.15 0.15 0.15 1.0]  GraphicEmissiveColor=[0.0 0.0 0.0 1.0]  GraphicShininess=75  DoExposeReferenceFrame=on  SerializedFrames=<Frames/>
      | Pièce CAO : Écrou de réglage 4.1 (RW-41_Ecrou-M6)
      | Masse 2.40 g : écrou hexagonal M6 en acier, 2,4 g.
      | Centre de masse et inertie : calculés sur la géométrie de la CAO.
  Écrou de réglage 4.2 : sm_lib/Body Elements/File Solid  Description=|  ExtGeomFileName=RW-41_Ecrou-M6.stl  UnitType=Custom  ExtGeomFileUnits=mm  StepReaderType=HEX  ExportConvexHullGeometry=off  InertiaType=Custom  BasedOnType=DensityFromFile  Density=1000  DensityUnits=kg/m^3  Mass=0.0024  MassUnits=kg  CenterOfMass=[1.6445434e-19 4.9031279e-19 -1.3524518e-36]  CenterOfMassUnits=m  MomentsOfInertia=[2.7128132e-08 2.7128132e-08 4.4256265e-08]  MomentsOfInertiaUnits=kg*m^2  ProductsOfInertia=[-1.5470275e-25 1.3498961e-25 -3.9289691e-24]  ProductsOfInertiaUnits=kg*m^2  GraphicType=FromGeometry  MarkerShape=Sphere  MarkerSize=10  GraphicVisPropType=SimpleVisualProperties  GraphicDiffuseColor=[0.788 0.635 0.153]  GraphicOpacity=1  GraphicSpecularColor=[0.5 0.5 0.5 1.0]  GraphicAmbientColor=[0.15 0.15 0.15 1.0]  GraphicEmissiveColor=[0.0 0.0 0.0 1.0]  GraphicShininess=75  DoExposeReferenceFrame=on  SerializedFrames=<Frames/>
      | Pièce CAO : Écrou de réglage 4.2 (RW-41_Ecrou-M6)
      | Masse 2.40 g : écrou hexagonal M6 en acier, 2,4 g.
      | Centre de masse et inertie : calculés sur la géométrie de la CAO.
  Écrou de serrage extérieur 1 : sm_lib/Body Elements/File Solid  Description=|  ExtGeomFileName=RW-41_Ecrou-M6.stl  UnitType=Custom  ExtGeomFileUnits=mm  StepReaderType=HEX  ExportConvexHullGeometry=off  InertiaType=Custom  BasedOnType=DensityFromFile  Density=1000  DensityUnits=kg/m^3  Mass=0.0024  MassUnits=kg  CenterOfMass=[1.6445434e-19 4.9031279e-19 -1.3524518e-36]  CenterOfMassUnits=m  MomentsOfInertia=[2.7128132e-08 2.7128132e-08 4.4256265e-08]  MomentsOfInertiaUnits=kg*m^2  ProductsOfInertia=[-1.5470275e-25 1.3498961e-25 -3.9289691e-24]  ProductsOfInertiaUnits=kg*m^2  GraphicType=FromGeometry  MarkerShape=Sphere  MarkerSize=10  GraphicVisPropType=SimpleVisualProperties  GraphicDiffuseColor=[0.788 0.635 0.153]  GraphicOpacity=1  GraphicSpecularColor=[0.5 0.5 0.5 1.0]  GraphicAmbientColor=[0.15 0.15 0.15 1.0]  GraphicEmissiveColor=[0.0 0.0 0.0 1.0]  GraphicShininess=75  DoExposeReferenceFrame=on  SerializedFrames=<Frames/>
      | Pièce CAO : Écrou de serrage extérieur 1 (RW-41_Ecrou-M6)
      | Masse 2.40 g : écrou hexagonal M6 en acier, 2,4 g.
      | Centre de masse et inertie : calculés sur la géométrie de la CAO.
  Écrou de serrage extérieur 2 : sm_lib/Body Elements/File Solid  Description=|  ExtGeomFileName=RW-41_Ecrou-M6.stl  UnitType=Custom  ExtGeomFileUnits=mm  StepReaderType=HEX  ExportConvexHullGeometry=off  InertiaType=Custom  BasedOnType=DensityFromFile  Density=1000  DensityUnits=kg/m^3  Mass=0.0024  MassUnits=kg  CenterOfMass=[1.6445434e-19 4.9031279e-19 -1.3524518e-36]  CenterOfMassUnits=m  MomentsOfInertia=[2.7128132e-08 2.7128132e-08 4.4256265e-08]  MomentsOfInertiaUnits=kg*m^2  ProductsOfInertia=[-1.5470275e-25 1.3498961e-25 -3.9289691e-24]  ProductsOfInertiaUnits=kg*m^2  GraphicType=FromGeometry  MarkerShape=Sphere  MarkerSize=10  GraphicVisPropType=SimpleVisualProperties  GraphicDiffuseColor=[0.788 0.635 0.153]  GraphicOpacity=1  GraphicSpecularColor=[0.5 0.5 0.5 1.0]  GraphicAmbientColor=[0.15 0.15 0.15 1.0]  GraphicEmissiveColor=[0.0 0.0 0.0 1.0]  GraphicShininess=75  DoExposeReferenceFrame=on  SerializedFrames=<Frames/>
      | Pièce CAO : Écrou de serrage extérieur 2 (RW-41_Ecrou-M6)
      | Masse 2.40 g : écrou hexagonal M6 en acier, 2,4 g.
      | Centre de masse et inertie : calculés sur la géométrie de la CAO.
  Écrou de serrage extérieur 3 : sm_lib/Body Elements/File Solid  Description=|  ExtGeomFileName=RW-41_Ecrou-M6.stl  UnitType=Custom  ExtGeomFileUnits=mm  StepReaderType=HEX  ExportConvexHullGeometry=off  InertiaType=Custom  BasedOnType=DensityFromFile  Density=1000  DensityUnits=kg/m^3  Mass=0.0024  MassUnits=kg  CenterOfMass=[1.6445434e-19 4.9031279e-19 -1.3524518e-36]  CenterOfMassUnits=m  MomentsOfInertia=[2.7128132e-08 2.7128132e-08 4.4256265e-08]  MomentsOfInertiaUnits=kg*m^2  ProductsOfInertia=[-1.5470275e-25 1.3498961e-25 -3.9289691e-24]  ProductsOfInertiaUnits=kg*m^2  GraphicType=FromGeometry  MarkerShape=Sphere  MarkerSize=10  GraphicVisPropType=SimpleVisualProperties  GraphicDiffuseColor=[0.788 0.635 0.153]  GraphicOpacity=1  GraphicSpecularColor=[0.5 0.5 0.5 1.0]  GraphicAmbientColor=[0.15 0.15 0.15 1.0]  GraphicEmissiveColor=[0.0 0.0 0.0 1.0]  GraphicShininess=75  DoExposeReferenceFrame=on  SerializedFrames=<Frames/>
      | Pièce CAO : Écrou de serrage extérieur 3 (RW-41_Ecrou-M6)
      | Masse 2.40 g : écrou hexagonal M6 en acier, 2,4 g.
      | Centre de masse et inertie : calculés sur la géométrie de la CAO.
  Écrou de serrage extérieur 4 : sm_lib/Body Elements/File Solid  Description=|  ExtGeomFileName=RW-41_Ecrou-M6.stl  UnitType=Custom  ExtGeomFileUnits=mm  StepReaderType=HEX  ExportConvexHullGeometry=off  InertiaType=Custom  BasedOnType=DensityFromFile  Density=1000  DensityUnits=kg/m^3  Mass=0.0024  MassUnits=kg  CenterOfMass=[1.6445434e-19 4.9031279e-19 -1.3524518e-36]  CenterOfMassUnits=m  MomentsOfInertia=[2.7128132e-08 2.7128132e-08 4.4256265e-08]  MomentsOfInertiaUnits=kg*m^2  ProductsOfInertia=[-1.5470275e-25 1.3498961e-25 -3.9289691e-24]  ProductsOfInertiaUnits=kg*m^2  GraphicType=FromGeometry  MarkerShape=Sphere  MarkerSize=10  GraphicVisPropType=SimpleVisualProperties  GraphicDiffuseColor=[0.788 0.635 0.153]  GraphicOpacity=1  GraphicSpecularColor=[0.5 0.5 0.5 1.0]  GraphicAmbientColor=[0.15 0.15 0.15 1.0]  GraphicEmissiveColor=[0.0 0.0 0.0 1.0]  GraphicShininess=75  DoExposeReferenceFrame=on  SerializedFrames=<Frames/>
      | Pièce CAO : Écrou de serrage extérieur 4 (RW-41_Ecrou-M6)
      | Masse 2.40 g : écrou hexagonal M6 en acier, 2,4 g.
      | Centre de masse et inertie : calculés sur la géométrie de la CAO.
  Écrou de serrage intérieur 1 : sm_lib/Body Elements/File Solid  Description=|  ExtGeomFileName=RW-41_Ecrou-M6.stl  UnitType=Custom  ExtGeomFileUnits=mm  StepReaderType=HEX  ExportConvexHullGeometry=off  InertiaType=Custom  BasedOnType=DensityFromFile  Density=1000  DensityUnits=kg/m^3  Mass=0.0024  MassUnits=kg  CenterOfMass=[1.6445434e-19 4.9031279e-19 -1.3524518e-36]  CenterOfMassUnits=m  MomentsOfInertia=[2.7128132e-08 2.7128132e-08 4.4256265e-08]  MomentsOfInertiaUnits=kg*m^2  ProductsOfInertia=[-1.5470275e-25 1.3498961e-25 -3.9289691e-24]  ProductsOfInertiaUnits=kg*m^2  GraphicType=FromGeometry  MarkerShape=Sphere  MarkerSize=10  GraphicVisPropType=SimpleVisualProperties  GraphicDiffuseColor=[0.788 0.635 0.153]  GraphicOpacity=1  GraphicSpecularColor=[0.5 0.5 0.5 1.0]  GraphicAmbientColor=[0.15 0.15 0.15 1.0]  GraphicEmissiveColor=[0.0 0.0 0.0 1.0]  GraphicShininess=75  DoExposeReferenceFrame=on  SerializedFrames=<Frames/>
      | Pièce CAO : Écrou de serrage intérieur 1 (RW-41_Ecrou-M6)
      | Masse 2.40 g : écrou hexagonal M6 en acier, 2,4 g.
      | Centre de masse et inertie : calculés sur la géométrie de la CAO.
  Écrou de serrage intérieur 2 : sm_lib/Body Elements/File Solid  Description=|  ExtGeomFileName=RW-41_Ecrou-M6.stl  UnitType=Custom  ExtGeomFileUnits=mm  StepReaderType=HEX  ExportConvexHullGeometry=off  InertiaType=Custom  BasedOnType=DensityFromFile  Density=1000  DensityUnits=kg/m^3  Mass=0.0024  MassUnits=kg  CenterOfMass=[1.6445434e-19 4.9031279e-19 -1.3524518e-36]  CenterOfMassUnits=m  MomentsOfInertia=[2.7128132e-08 2.7128132e-08 4.4256265e-08]  MomentsOfInertiaUnits=kg*m^2  ProductsOfInertia=[-1.5470275e-25 1.3498961e-25 -3.9289691e-24]  ProductsOfInertiaUnits=kg*m^2  GraphicType=FromGeometry  MarkerShape=Sphere  MarkerSize=10  GraphicVisPropType=SimpleVisualProperties  GraphicDiffuseColor=[0.788 0.635 0.153]  GraphicOpacity=1  GraphicSpecularColor=[0.5 0.5 0.5 1.0]  GraphicAmbientColor=[0.15 0.15 0.15 1.0]  GraphicEmissiveColor=[0.0 0.0 0.0 1.0]  GraphicShininess=75  DoExposeReferenceFrame=on  SerializedFrames=<Frames/>
      | Pièce CAO : Écrou de serrage intérieur 2 (RW-41_Ecrou-M6)
      | Masse 2.40 g : écrou hexagonal M6 en acier, 2,4 g.
      | Centre de masse et inertie : calculés sur la géométrie de la CAO.
  Écrou de serrage intérieur 3 : sm_lib/Body Elements/File Solid  Description=|  ExtGeomFileName=RW-41_Ecrou-M6.stl  UnitType=Custom  ExtGeomFileUnits=mm  StepReaderType=HEX  ExportConvexHullGeometry=off  InertiaType=Custom  BasedOnType=DensityFromFile  Density=1000  DensityUnits=kg/m^3  Mass=0.0024  MassUnits=kg  CenterOfMass=[1.6445434e-19 4.9031279e-19 -1.3524518e-36]  CenterOfMassUnits=m  MomentsOfInertia=[2.7128132e-08 2.7128132e-08 4.4256265e-08]  MomentsOfInertiaUnits=kg*m^2  ProductsOfInertia=[-1.5470275e-25 1.3498961e-25 -3.9289691e-24]  ProductsOfInertiaUnits=kg*m^2  GraphicType=FromGeometry  MarkerShape=Sphere  MarkerSize=10  GraphicVisPropType=SimpleVisualProperties  GraphicDiffuseColor=[0.788 0.635 0.153]  GraphicOpacity=1  GraphicSpecularColor=[0.5 0.5 0.5 1.0]  GraphicAmbientColor=[0.15 0.15 0.15 1.0]  GraphicEmissiveColor=[0.0 0.0 0.0 1.0]  GraphicShininess=75  DoExposeReferenceFrame=on  SerializedFrames=<Frames/>
      | Pièce CAO : Écrou de serrage intérieur 3 (RW-41_Ecrou-M6)
      | Masse 2.40 g : écrou hexagonal M6 en acier, 2,4 g.
      | Centre de masse et inertie : calculés sur la géométrie de la CAO.
  Écrou de serrage intérieur 4 : sm_lib/Body Elements/File Solid  Description=|  ExtGeomFileName=RW-41_Ecrou-M6.stl  UnitType=Custom  ExtGeomFileUnits=mm  StepReaderType=HEX  ExportConvexHullGeometry=off  InertiaType=Custom  BasedOnType=DensityFromFile  Density=1000  DensityUnits=kg/m^3  Mass=0.0024  MassUnits=kg  CenterOfMass=[1.6445434e-19 4.9031279e-19 -1.3524518e-36]  CenterOfMassUnits=m  MomentsOfInertia=[2.7128132e-08 2.7128132e-08 4.4256265e-08]  MomentsOfInertiaUnits=kg*m^2  ProductsOfInertia=[-1.5470275e-25 1.3498961e-25 -3.9289691e-24]  ProductsOfInertiaUnits=kg*m^2  GraphicType=FromGeometry  MarkerShape=Sphere  MarkerSize=10  GraphicVisPropType=SimpleVisualProperties  GraphicDiffuseColor=[0.788 0.635 0.153]  GraphicOpacity=1  GraphicSpecularColor=[0.5 0.5 0.5 1.0]  GraphicAmbientColor=[0.15 0.15 0.15 1.0]  GraphicEmissiveColor=[0.0 0.0 0.0 1.0]  GraphicShininess=75  DoExposeReferenceFrame=on  SerializedFrames=<Frames/>
      | Pièce CAO : Écrou de serrage intérieur 4 (RW-41_Ecrou-M6)
      | Masse 2.40 g : écrou hexagonal M6 en acier, 2,4 g.
      | Centre de masse et inertie : calculés sur la géométrie de la CAO.
  F : PMIOPort  Side=Left
  connections:
  RW-50_Fils-moteur/RConn1 -- F/RConn1 -- RW-51_Fils-alim-ESC/RConn1 -- RW-52_Cable-alimentation/RConn1 -- RW-53_Cables-commande-ESC/RConn1 -- RW-54_Cables-capteurs/RConn1 -- RW-55_Cable-BNO055/RConn1 -- RW-56_Nappe-signaux/RConn1 -- Corps central/RConn1 -- Plateau/RConn1 -- Bornier/RConn1 -- Pose BNO055/LConn1 -- Pose Barrette 1/LConn1 -- Pose Barrette 2/LConn1 -- Pose ESC 1/LConn1 -- Pose ESC 2/LConn1 -- Pose ESC 3/LConn1 -- Pose ESC 4/LConn1 -- Pose Entretoise de la carte 1/LConn1 -- Pose Entretoise de la carte 2/LConn1 -- Pose Entretoise de la carte 3/LConn1 -- Pose Entretoise de la carte 4/LConn1 -- Pose Carte de distribution XT60/LConn1 -- Pose Fiche XT60 de l'ESC 1/LConn1 -- Pose Fiche XT60 de l'ESC 2/LConn1 -- Pose Fiche XT60 de l'ESC 3/LConn1 -- Pose Fiche XT60 de l'ESC 4/LConn1 -- Pose Fiche XT60 de l'alimentation/LConn1 -- Pose Tige d'équilibrage 1/LConn1 -- Pose Écrou de serrage intérieur 1/LConn1 -- Pose Écrou de serrage extérieur 1/LConn1 -- Pose Écrou de réglage 1.1/LConn1 -- Pose Écrou de réglage 1.2/LConn1 -- Pose Écrou de réglage 1.3/LConn1 -- Pose Tige d'équilibrage 2/LConn1 -- Pose Écrou de serrage intérieur 2/LConn1 -- Pose Écrou de serrage extérieur 2/LConn1 -- Pose Écrou de réglage 2.1/LConn1 -- Pose Tige d'équilibrage 3/LConn1 -- Pose Écrou de serrage intérieur 3/LConn1 -- Pose Écrou de serrage extérieur 3/LConn1 -- Pose Tige d'équilibrage 4/LConn1 -- Pose Écrou de serrage intérieur 4/LConn1 -- Pose Écrou de serrage extérieur 4/LConn1 -- Pose Écrou de réglage 4.1/LConn1 -- Pose Écrou de réglage 4.2/LConn1
  Pose BNO055/RConn1 -- BNO055/RConn1
  Pose Barrette 1/RConn1 -- Barrette 1/RConn1
  Pose Barrette 2/RConn1 -- Barrette 2/RConn1
  Pose ESC 1/RConn1 -- ESC 1/RConn1
  Pose ESC 2/RConn1 -- ESC 2/RConn1
  Pose ESC 3/RConn1 -- ESC 3/RConn1
  Pose ESC 4/RConn1 -- ESC 4/RConn1
  Pose Entretoise de la carte 1/RConn1 -- Entretoise de la carte 1/RConn1
  Pose Entretoise de la carte 2/RConn1 -- Entretoise de la carte 2/RConn1
  Pose Entretoise de la carte 3/RConn1 -- Entretoise de la carte 3/RConn1
  Pose Entretoise de la carte 4/RConn1 -- Entretoise de la carte 4/RConn1
  Pose Carte de distribution XT60/RConn1 -- Carte de distribution XT60/RConn1
  Pose Fiche XT60 de l'ESC 1/RConn1 -- Fiche XT60 de l'ESC 1/RConn1
  Pose Fiche XT60 de l'ESC 2/RConn1 -- Fiche XT60 de l'ESC 2/RConn1
  Pose Fiche XT60 de l'ESC 3/RConn1 -- Fiche XT60 de l'ESC 3/RConn1
  Pose Fiche XT60 de l'ESC 4/RConn1 -- Fiche XT60 de l'ESC 4/RConn1
  Pose Fiche XT60 de l'alimentation/RConn1 -- Fiche XT60 de l'alimentation/RConn1
  Pose Tige d'équilibrage 1/RConn1 -- Tige d'équilibrage 1/RConn1
  Pose Écrou de serrage intérieur 1/RConn1 -- Écrou de serrage intérieur 1/RConn1
  Pose Écrou de serrage extérieur 1/RConn1 -- Écrou de serrage extérieur 1/RConn1
  Pose Écrou de réglage 1.1/RConn1 -- Écrou de réglage 1.1/RConn1
  Pose Écrou de réglage 1.2/RConn1 -- Écrou de réglage 1.2/RConn1
  Pose Écrou de réglage 1.3/RConn1 -- Écrou de réglage 1.3/RConn1
  Pose Tige d'équilibrage 2/RConn1 -- Tige d'équilibrage 2/RConn1
  Pose Écrou de serrage intérieur 2/RConn1 -- Écrou de serrage intérieur 2/RConn1
  Pose Écrou de serrage extérieur 2/RConn1 -- Écrou de serrage extérieur 2/RConn1
  Pose Écrou de réglage 2.1/RConn1 -- Écrou de réglage 2.1/RConn1
  Pose Tige d'équilibrage 3/RConn1 -- Tige d'équilibrage 3/RConn1
  Pose Écrou de serrage intérieur 3/RConn1 -- Écrou de serrage intérieur 3/RConn1
  Pose Écrou de serrage extérieur 3/RConn1 -- Écrou de serrage extérieur 3/RConn1
  Pose Tige d'équilibrage 4/RConn1 -- Tige d'équilibrage 4/RConn1
  Pose Écrou de serrage intérieur 4/RConn1 -- Écrou de serrage intérieur 4/RConn1
  Pose Écrou de serrage extérieur 4/RConn1 -- Écrou de serrage extérieur 4/RConn1
  Pose Écrou de réglage 4.1/RConn1 -- Écrou de réglage 4.1/RConn1
  Pose Écrou de réglage 4.2/RConn1 -- Écrou de réglage 4.2/RConn1
